simulink model "Particle_swarm_based_PV_MPPT"  (R2017a)
(part 3 of 6)

      mask TypeOptions ModuleName: User-defined | 1Soltech 1STH-215-P | 1Soltech 1STH-220-P | 1Soltech 1STH-225-P | 1Soltech 1STH-230-P | 1Soltech 1STH-235-WH | 1Soltech 1STH-240-WH | 1Soltech 1STH-245-WH | 1Soltech 1STH-FRL-4H-245-M60-BLK | 1Soltech 1STH-250-WH | 1Soltech 1STH-FRL-4H-250-M60-BLK | 1Soltech 1STH-FRL-4H-255-M60-BLK | 1Soltech 1STH-FRL-4H-260-M60-BLK | 1Soltech 1STH-335-WH | 1Soltech 1STH-340-WH | 1Soltech 1STH-345-WH | 1Soltech 1STH-350-WH | A10Green Technology A10J-S72-175 | A10Green Technology A10J-S72-180 | A10Green Technology A10J-S72-185 | A10Green Technology A10J-M60-220 | A10Green Technology A10J-M60-225 | A10Green Technology A10J-M60-230 | A10Green Technology A10J-M60-235 | A10Green Technology A10J-M60-240 | A2Peak Power POWER ON P220-6x10 | Aavid Solar ASMS-165P | Aavid Solar ASMS-180M | Aavid Solar ASMS-185M | Aavid Solar ASMS-220P | Aavid Solar ASMS-225M | Aavid Solar ASMS-230P | Aavid Solar ASMS-235M | Aavid Solar ASMS-270P | Aavid Thermalloy ASMP-175M | Aavid Thermalloy ASMP-180M | AblyTek 5MN6C175-A0 | AblyTek 5MN6C180-A0 | AblyTek 5MN6C185-A0 | AblyTek 6PN6A220-A0 | AblyTek 6PN6A225-A0 | AblyTek 6PN6A230-A0 | AblyTek 6PN6A235-A0 | AblyTek 6PN6A240-A0 | AccuSolar Power ASP610-B230 | Advance Solar Hydro Wind Power API-150 | Advance Solar Hydro Wind Power API-160 | Advance Solar Hydro Wind Power API-165 | Advance Solar Hydro Wind Power API-170 | Advance Solar Hydro Wind Power API-175 | Advance Solar Hydro Wind Power API-180 | Advance Solar Hydro Wind Power API156P-200 | Advance Solar Hydro Wind Power API156P-210 | Advance Solar Hydro Wind Power API156P-220 | Advance Solar Hydro Wind Power API156P-230 | Advanced Renewable Energy AREi-210W-M6-G | Advanced Renewable Energy AREi-215W-M6-G | Advanced Renewable Energy AREi-220W-M6-G | Advanced Renewable Energy AREi-225W-M6-G | Advanced Renewable Energy AREi-230W-M6-G | aleo solar S16.165 | aleo solar S16.170 | aleo solar S16.175 | aleo solar S16.180 | aleo solar S16.185 | aleo solar A18.210 | Aleo Solar A18U210 ulr | aleo solar S18.210 | Aleo Solar S18U210 ulr | aleo solar A18.215 | Aleo Solar A18U215 ulr | aleo solar S18.215 | Aleo Solar S18U215 ulr | aleo solar A18.220 | Aleo Solar A18U220 ulr | aleo solar S18.220 | Aleo Solar S18U220 ulr | aleo solar A18.225 | Aleo Solar A18U225 ulr | aleo solar S18.225 | Aleo Solar S18U225 ulr | aleo solar A18.230 | Aleo Solar A18U230 ulr | aleo solar A79.230 | Aleo Solar A79U230 ulr | aleo solar S18.230 | Aleo Solar S18U230 ulr | aleo solar S79.230 | Aleo Solar S79U230 ulr | aleo solar A18.235 | Aleo Solar A18U235 ulr | aleo solar A79.235 | Aleo Solar A79U235 ulr | aleo solar S18.235 | Aleo Solar S18U235 ulr | Aleo Solar S19U235 ulr | aleo solar S79.235 | Aleo Solar S79U235 ulr | aleo solar A18.240 | Aleo Solar A18U240 ulr | aleo solar A79.240 | Aleo Solar A79U240 ulr | aleo solar S18.240 | Aleo Solar S18U240 | Aleo Solar S18U240 ulr | Aleo Solar S19U240 ulr | aleo solar S79.240 | Aleo Solar S79U240 ulr | aleo solar A18.245 | Aleo Solar A18U245 ulr | aleo solar A79.245 | Aleo Solar A79U245 ulr | aleo solar S18.245 | Aleo Solar S18U245 | Aleo Solar S18U245 ulr | Aleo Solar S19U245 ulr | aleo solar S79.245 | Aleo Solar S79U245 ulr | aleo solar A79.250 | Aleo Solar A79U250 ulr | Aleo Solar S18U250 | Aleo Solar S19H250 | Aleo Solar S19U250 ulr | aleo solar S79.250 | Aleo Solar S79U250 | Aleo Solar S79U250 ulr | Aleo Solar S18U255 | Aleo Solar S19H255 | Aleo Solar S19U255 ulr | Aleo Solar S79U255 | Aleo Solar S18U260 | Aleo Solar S19H260 | Aleo Solar S79U260 | Aleo Solar S19H265 | Aleo Solar S79U265 | Aleo Solar S19H270 | Aleo Solar S79U270 | alfasolar alfasolar P6L60-220 | alfasolar alfasolar P6L60-225 | alfasolar alfasolar P6L60-230 | alfasolar alfasolar P6L60-235 | alfasolar alfasolar M6L60-240 | alfasolar alfasolar P6L60-240 | alfasolar alfasolar M6L60-245 | alfasolar alfasolar P6L60-245 | alfasolar alfasolar M6L60-250 | alfasolar alfasolar P6L60-250 | alfasolar alfasolar M6L60-255 | alfasolar alfasolar M6L60-260 | alfasolar alfasolar M6L60-265 | Alps Technology ATI-S572-175 | Alps Technology ATI-S572-180 | Alps Technology ATI-S572-185 | Alps Technology ATI-M660-220 | Alps Technology ATI-M660-225 | Alps Technology ATI-M660-230 | Alps Technology ATI-M660-235 | Alps Technology ATI-M660-240 | American Choice Solar ACS-215-P | American Choice Solar ACS-220-P | American Choice Solar ACS-225-P | American Choice Solar ACS-230-P | American Choice Solar ACS-235-M | American Choice Solar ACS-240-M | American Choice Solar ACS-245-M | American Choice Solar ACS-250-M | American Choice Solar ACS-335-M | American Solar Wholesale ASW-175M | American Solar Wholesale ASW-180M | American Solar Wholesale ASW-185M | American Solar Wholesale ASW-215P | American Solar Wholesale ASW-220P | American Solar Wholesale ASW-225M | American Solar Wholesale ASW-225P | American Solar Wholesale ASW-230M | American Solar Wholesale ASW-230P | American Solar Wholesale ASW-235M | American Solar Wholesale ASW-235P | American Solar Wholesale ASW-240M-60 | American Solar Wholesale ASW-245M | American Solar Wholesale ASW-250P | American Solar Wholesale ASW-260M | American Solar Wholesale ASW-260P | American Solar Wholesale ASW-265M | American Solar Wholesale ASW-270M | American Solar Wholesale ASW-270P | American Solar Wholesale ASW-275M | American Solar Wholesale ASW-280M | American Value SM240-5M | American Value SM245-5M | American Value SM250-5M | American Value SM255-5M | American Value SM260-5M | Andalay Solar ST_165_1_DC0_0_B | Andalay Solar ST165-1 | Andalay Solar ST_170_1_DC0_0_B | Andalay Solar ST170-1 | Andalay Solar ST_175_1_DC0_0_B | Andalay Solar ST175-1 | Andalay Solar ST-175-1AC1-A-A | Andalay Solar ST-175-1AC3-B-A | Andalay Solar KC180-1 | Andalay Solar ST_180_1_DC0_0_B | Andalay Solar ST180-1 | Andalay Solar ST_185_1_DC0_0_B | Andalay Solar ST-185-1 | Andalay Solar ST-185-1AC1-A-A | Andalay Solar ST-185-1AC1-A-B | Andalay Solar ST-185-1AC3-B-A | Andalay Solar ST-185-1AC3-B-B | Andalay Solar ST_190_1_DC0_0_B | Andalay Solar ST-190-1AC1-A-B | Andalay Solar ST-190-1AC3-B-B | Andalay Solar ST_195_1_DC0_0_B | Andalay Solar ST-195-1AC1-A-B | Andalay Solar ST-195-1AC3-B-B | Andalay Solar KC205-1 | Andalay Solar KC210-1 | Andalay Solar LW-230-1-AC0-D-B | Andalay Solar LW-230-1-AC1-A-B | Andalay Solar LW-230-1-AC2-D-B | Andalay Solar LW-230-1-AC3-B-B | Andalay Solar LW-230-1-DC0-0-B | Andalay Solar LW-230-1-DC0-0-BL | Andalay Solar LW-230-1-DC1-0-B | Andalay Solar LW-235-1-AC0-D-B | Andalay Solar LW-235-1-AC1-A-B | Andalay Solar LW-235-1-AC2-D-B | Andalay Solar LW-235-1-AC3-B-B | Andalay Solar LW-235-1-DC0-0-B | Andalay Solar LW-235-1-DC0-0-BL | Andalay Solar LW-235-1-DC1-0-B | Andalay Solar LW-240-1-AC0-D-B | Andalay Solar LW-240-1-AC1-A-B | Andalay Solar LW-240-1-AC2-D-B | Andalay Solar LW-240-1-AC3-B-B | Andalay Solar LW-240-1-DC0-0-B | Andalay Solar LW-240-1-DC0-0-BL | Andalay Solar LW-240-1-DC1-0-B | Andalay Solar TW-240-1-AC2-D-B | Andalay Solar TW-240-1-DC4-0-B | Andalay Solar TW-245-1-AC2-D-B | Andalay Solar TW-245-1-DC4-0-B | Andalay Solar TW-250-1-AC2-D-B | Andalay Solar TW-250-1-DC4-0-B | Andalay Solar ST_260_1_DC0_0_B | Andalay Solar ST_270_1_DC0_0_B | Andalay Solar ST_280_1_DC0_0_B | Andalay Solar ST_290_1_DC0_0_B | Anji Dasol Solar Energy Science & Technology DS-A4-210 | Anji Dasol Solar Energy Science & Technology DS-A4-215 | Anji Dasol Solar Energy Science & Technology DS-A4-220 | Anji Dasol Solar Energy Science & Technology DS-A4-225 | Anji Dasol Solar Energy Science & Technology DS-A4-230 | Anji Technology AJP-S572-175 | Anji Technology AJP-S572-180 | Anji Technology AJP-S572-185 | Anji Technology AJP-M660-220 | Anji Technology AJP-M660-225 | Anji Technology AJP-M660-230 | Anji Technology AJP-M660-235 | Anji Technology AJP-M660-240 | Anji Technology AJP-M660-245 | Anji Technology AJP-M660-250 | Antaris Solar AS P 230 | Antaris Solar SM-230PC8 | Antaris Solar SM-235PC8 | Antaris Solar SM-240PC8 | Antaris Solar SM-245PC8 | Antaris Solar SM-250PC8 | Antaris Solar SM-275PC8 | Antaris Solar SM-280PC8 | Antaris Solar SM-285PC8 | Antaris Solar SM-290PC8 | Antaris Solar SM-295PC8 | Apollo Solar Energy ASEC-120G6M | Apollo Solar Energy ASEC-125G6M | Apollo Solar Energy ASEC-125G6S | Apollo Solar Energy ASEC-130G6M | Apollo Solar Energy ASEC-130G6S | Apollo Solar Energy ASEC-135G6M | Apollo Solar Energy ASEC-135G6S | Apollo Solar Energy ASEC-140G6M | Apollo Solar Energy ASEC-140G6S | Apollo Solar Energy ASEC-145G6M49 | Apollo Solar Energy ASEC-145G6S49 | Apollo Solar Energy ASEC-150G6M49 | Apollo Solar Energy ASEC-150G6S49 | Apollo Solar Energy ASEC-155G6M49 | Apollo Solar Energy ASEC-155G6S49 | Apollo Solar Energy ASEC-175G6M | Apollo Solar Energy ASEC-175G6S | Apollo Solar Energy ASEC-180G6M | Apollo Solar Energy ASEC-180G6S | Apollo Solar Energy ASEC-185G6M | Apollo Solar Energy ASEC-185G6S | Apollo Solar Energy ASEC-190G6M | Apollo Solar Energy ASEC-190G6M68 | Apollo Solar Energy ASEC-190G6S | Apollo Solar Energy ASEC-190G6S68 | Apollo Solar Energy ASEC-195G6M | Apollo Solar Energy ASEC-195G6M68 | Apollo Solar Energy ASEC-195G6S | Apollo Solar Energy ASEC-195G6S68 | Apollo Solar Energy ASEC-200G6M | Apollo Solar Energy ASEC-200G6M68 | Apollo Solar Energy ASEC-200G6S | Apollo Solar Energy ASEC-200G6S68 | Apollo Solar Energy ASEC-205G6M | Apollo Solar Energy ASEC-205G6M68 | Apollo Solar Energy ASEC-205G6S | Apollo Solar Energy ASEC-205G6S68 | Apollo Solar Energy ASEC-210G6M | Apollo Solar Energy ASEC-210G6M68 | Apollo Solar Energy ASEC-210G6S | Apollo Solar Energy ASEC-210G6S68 | Apollo Solar Energy ASEC-215G6M | Apollo Solar Energy ASEC-215G6M68 | Apollo Solar Energy ASEC-215G6M69 | Apollo Solar Energy ASEC-215G6S | Apollo Solar Energy ASEC-215G6S68 | Apollo Solar Energy ASEC-215G6S69 | Apollo Solar Energy ASEC-220G6M | Apollo Solar Energy ASEC-220G6M68 | Apollo Solar Energy ASEC-220G6M69 | Apollo Solar Energy ASEC-220G6S | Apollo Solar Energy ASEC-220G6S68 | Apollo Solar Energy ASEC-220G6S69 | Apollo Solar Energy ASEC-225G6M | Apollo Solar Energy ASEC-225G6M69 | Apollo Solar Energy ASEC-225G6S | Apollo Solar Energy ASEC-225G6S69 | Apollo Solar Energy ASEC-230G6M | Apollo Solar Energy ASEC-230G6M69 | Apollo Solar Energy ASEC-230G6S | Apollo Solar Energy ASEC-230G6S69 | Apollo Solar Energy ASEC-235G6M | Apollo Solar Energy ASEC-235G6M69 | Apollo Solar Energy ASEC-235G6S | Apollo Solar Energy ASEC-235G6S69 | Apollo Solar Energy ASEC-240G6M69 | Apollo Solar Energy ASEC-240G6M6A | Apollo Solar Energy ASEC-240G6S69 | Apollo Solar Energy ASEC-240G6S6A | Apollo Solar Energy ASEC-245G6M | Apollo Solar Energy ASEC-245G6M69 | Apollo Solar Energy ASEC-245G6M6A | Apollo Solar Energy ASEC-245G6S69 | Apollo Solar Energy ASEC-245G6S6A | Apollo Solar Energy ASEC-250G6M | Apollo Solar Energy ASEC-250G6M6A | Apollo Solar Energy ASEC-250G6M6B | Apollo Solar Energy ASEC-250G6S6A | Apollo Solar Energy ASEC-250G6S6B | Apollo Solar Energy ASEC-255G6M | Apollo Solar Energy ASEC-255G6M6A | Apollo Solar Energy ASEC-255G6M6B | Apollo Solar Energy ASEC-255G6S | Apollo Solar Energy ASEC-255G6S6A | Apollo Solar Energy ASEC-255G6S6B | Apollo Solar Energy ASEC-260G6M | Apollo Solar Energy ASEC-260G6M6A | Apollo Solar Energy ASEC-260G6M6B | Apollo Solar Energy ASEC-260G6S | Apollo Solar Energy ASEC-260G6S6A | Apollo Solar Energy ASEC-260G6S6B | Apollo Solar Energy ASEC-265G6M | Apollo Solar Energy ASEC-265G6M6A | Apollo Solar Energy ASEC-265G6M6B | Apollo Solar Energy ASEC-265G6S | Apollo Solar Energy ASEC-265G6S6A | Apollo Solar Energy ASEC-265G6S6B | Apollo Solar Energy ASEC-270G6M | Apollo Solar Energy ASEC-270G6M6A | Apollo Solar Energy ASEC-270G6M6B | Apollo Solar Energy ASEC-270G6S | Apollo Solar Energy ASEC-270G6S6A | Apollo Solar Energy ASEC-270G6S6B | Apollo Solar Energy ASEC-275G6M | Apollo Solar Energy ASEC-275G6M6B | Apollo Solar Energy ASEC-275G6S | Apollo Solar Energy ASEC-275G6S6B | Apollo Solar Energy ASEC-280G6M | Apollo Solar Energy ASEC-280G6M6B | Apollo Solar Energy ASEC-280G6S | Apollo Solar Energy ASEC-280G6S6B | Apollo Solar Energy ASEC-285G6M | Apollo Solar Energy ASEC-285G6M6B | Apollo Solar Energy ASEC-285G6S | Apollo Solar Energy ASEC-285G6S6B | Apollo Solar Energy ASEC-290G6M | Apollo Solar Energy ASEC-290G6M6B | Apollo Solar Energy ASEC-290G6S | Apollo Solar Energy ASEC-290G6S6B | Apollo Solar Energy ASEC-295G6M | Apollo Solar Energy ASEC-295G6M6B | Apollo Solar Energy ASEC-295G6S | Apollo Solar Energy ASEC-295G6S6B | Apollo Solar Energy ASEC-300G6M | Apollo Solar Energy ASEC-300G6S | Apollo Solar Energy ASEC-305G6M | Apollo Solar Energy ASEC-305G6S | Apollo Solar Energy ASEC-310G6M | Apollo Solar Energy ASEC-310G6S | Apollo Solar Energy ASEC-315G6M | Apollo Solar Energy ASEC-315G6S | Apollo Solar Energy ASEC-320G6M | Apollo Solar Energy ASEC-320G6S | Apollo Solar Energy ASEC-325G6M | Apollo Solar Energy ASEC-325G6S | APOS Energy AP130 | APOS Energy AP135 | APOS Energy AS135 | APOS Energy AP140 | APOS Energy AS140 | APOS Energy AS145 | APOS Energy AP175 | APOS Energy AP180 | APOS Energy AS180 | APOS Energy AP185 | APOS Energy AS185 | APOS Energy AP190 | APOS Energy AS190 | APOS Energy AP195 | APOS Energy AS195 | APOS Energy AP 200M | APOS Energy AP200 | APOS Energy AS200 | APOS Energy AP 205M | APOS Energy AP205 | APOS Energy AS205 | APOS Energy AP 210M | APOS Energy AP210 | APOS Energy AS210 | APOS Energy AP 215M | APOS Energy AP215 | APOS Energy AS215 | APOS Energy AP 220M | APOS Energy AP220 | APOS Energy AS220 | APOS Energy AP 225M | APOS Energy AP225 | APOS Energy AS225 | APOS Energy AP 230M | APOS Energy AP230 | APOS Energy AS230 | APOS Energy AP 235M | APOS Energy AS235 | APOS Energy AP 240M | APOS Energy AS240 | Applied Quantum Technology AQT125MA-160W | Applied Quantum Technology AQT125MA-165W | Applied Quantum Technology AQT125MA-170W | Applied Quantum Technology AQT125MA-175W | Applied Quantum Technology AQT125MA-180W | Applied Quantum Technology AQT156PA-190W | Applied Quantum Technology AQT156PA-195W | Applied Quantum Technology AQT156PA-200W | Applied Quantum Technology AQT156PA-205W | Applied Quantum Technology AQT156PA-210W | Applied Quantum Technology AQT156PA-215W | Applied Quantum Technology AQT156PA-220W | Applied Quantum Technology AQT156PA-225W | Applied Quantum Technology AQT156PA-230W | Armageddon Energy SolarClover Dual Module | ASUN Energy ASM190PCA0G101 | ASUN Energy ASM195PCA0G101 | ASUN Energy ASM200PCA0G101 | ASUN Energy ASM205PCA0G101 | ASUN Energy ASM210PCA0G101 | Atersa (Aplicaciones Tecnicas de la Energia) A-225P | Atersa (Aplicaciones Tecnicas de la Energia) A-230P | Atersa (Aplicaciones Tecnicas de la Energia) A-235P | Atersa (Aplicaciones Tecnicas de la Energia) A-240P | Atersa (Aplicaciones Tecnicas de la Energia) A-245P | Atersa (Aplicaciones Tecnicas de la Energia) A-250P | Atersa (Aplicaciones Tecnicas de la Energia) A-275P | Atersa (Aplicaciones Tecnicas de la Energia) A-280P | Atersa (Aplicaciones Tecnicas de la Energia) A-285P | Atersa (Aplicaciones Tecnicas de la Energia) A-290P | Atersa (Aplicaciones Tecnicas de la Energia) A-295P | Atersa (Aplicaciones Tecnicas de la Energia) A-300P | Atlantis Energy Systems SS125LM | Atlantis Energy Systems SS156LM | Atlantis Energy Systems TS125LM | Atlantis Energy Systems TSG156LM | Atlantis Energy Systems TSG156GM | Atlantis Energy Systems SS125GM | Atlantis Energy Systems SS156GM | Atlantis Energy Systems TS125GM | Atlantis Energy AES-SS-100-C | Atlantis Energy AES-SS-100-W | AU Optronics PM180M00.0_170 | AU Optronics PM180M00.0_175 | AU Optronics PM180M00.0_180 | AU Optronics PM200M00_190 | AU Optronics PM200M00_195 | AU Optronics PM200M00_200 | AU Optronics PM200M00_205 | AU Optronics PM200M00_210 | AU Optronics PM220P00_215 | AU Optronics PM220P02.0_215 | AU Optronics PM220P00.4_220 | AU Optronics PM220P00_220 | AU Optronics PM220P01.0_220 | AU Optronics PM220P02.0_220 | AU Optronics PM220P00.4_225 | AU Optronics PM220P00_225 | AU Optronics PM220P01.0_225 | AU Optronics PM220P02.0_225 | AU Optronics PM245P00_225 | AU Optronics PM220P00.4_230 | AU Optronics PM220P00_230 | AU Optronics PM220P01.0_230 | AU Optronics PM220P02.0_230 | AU Optronics PM240P00_230 | AU Optronics PM245P00_230 | AU Optronics PM245P01_230 | AU Optronics PM060PA0_235 | AU Optronics PM060PA1_235 | AU Optronics PM060PA2_235 | AU Optronics PM220P00.4_235 | AU Optronics PM220P00_235 | AU Optronics PM220P01.0_235 | AU Optronics PM240P00_235 | AU Optronics PM240PA0_235 | AU Optronics PM245P00_235 | AU Optronics PM245P01_235 | AU Optronics PM245PA0_235 | AU Optronics PM245PA1_235 | AU Optronics PM245PA2_235 | AU Optronics PM060MA0_240 | AU Optronics PM060MA1_240 | AU Optronics PM060MA2_240 | AU Optronics PM060PA0_240 | AU Optronics PM060PA1_240 | AU Optronics PM060PA2_240 | AU Optronics PM220P01.0_240 | AU Optronics PM240P00_240 | AU Optronics PM240PA0_240 | AU Optronics PM245P00_240 | AU Optronics PM245P01_240 | AU Optronics PM245PA0_240 | AU Optronics PM245PA1_240 | AU Optronics PM245PA2_240 | AU Optronics PM250M00_240 | AU Optronics PM250M02_240 | AU Optronics PM250MA0_240 | AU Optronics PM250MA1_240 | AU Optronics PM250MA2_240 | AU Optronics PM060MA0_245 | AU Optronics PM060MA1_245 | AU Optronics PM060MA2_245 | AU Optronics PM060PA0_245 | AU Optronics PM060PA1_245 | AU Optronics PM060PA2_245 | AU Optronics PM240P00_245 | AU Optronics PM240PA0_245 | AU Optronics PM245P00_245 | AU Optronics PM245P01_245 | AU Optronics PM245PA0_245 | AU Optronics PM245PA1_245 | AU Optronics PM245PA2_245 | AU Optronics PM250M00_245 | AU Optronics PM250MA0_245 | AU Optronics PM250MA1_245 | AU Optronics PM250MA2_245 | AU Optronics PM060MA0_250 | AU Optronics PM060MA1_250 | AU Optronics PM060MA2_250 | AU Optronics PM060PA0_250 | AU Optronics PM060PA1_250 | AU Optronics PM060PA2_250 | AU Optronics PM245P00_250 | AU Optronics PM245P01_250 | AU Optronics PM245PA0_250 | AU Optronics PM245PA1_250 | AU Optronics PM245PA2_250 | AU Optronics PM250M00_250 | AU Optronics PM250M01_250 | AU Optronics PM250MA0_250 | AU Optronics PM250MA1_250 | AU Optronics PM250MA2_250 | AU Optronics PM060MA0_255 | AU Optronics PM060MA1_255 | AU Optronics PM060MA2_255 | AU Optronics PM060PA0_255 | AU Optronics PM060PA1_255 | AU Optronics PM060PA2_255 | AU Optronics PM245P00_255 | AU Optronics PM245P01_255 | AU Optronics PM245PA0_255 | AU Optronics PM245PA1_255 | AU Optronics PM245PA2_255 | AU Optronics PM250M00_255 | AU Optronics PM250M01_255 | AU Optronics PM250MA0_255 | AU Optronics PM250MA1_255 | AU Optronics PM250MA2_255 | AU Optronics PM060MA0_260 | AU Optronics PM060MA1_260 | AU Optronics PM060MA2_260 | AU Optronics PM060PA0_260 | AU Optronics PM060PA1_260 | AU Optronics PM060PA2_260 | AU Optronics PM245P00_260 | AU Optronics PM245P01_260 | AU Optronics PM245PA0_260 | AU Optronics PM245PA1_260 | AU Optronics PM245PA2_260 | AU Optronics PM250M00_260 | AU Optronics PM250M01_260 | AU Optronics PM250MA0_260 | AU Optronics PM250MA1_260 | AU Optronics PM250MA2_260 | AU Optronics PM060MA0_265 | AU Optronics PM060MA1_265 | AU Optronics PM060MA2_265 | AU Optronics PM250M00_265 | AU Optronics PM250M01_265 | AU Optronics PM250MA0_265 | AU Optronics PM250MA1_265 | AU Optronics PM250MA2_265 | AU Optronics PM060MA0_270 | AU Optronics PM060MA1_270 | AU Optronics PM060MA2_270 | AU Optronics PM250M00_270 | AU Optronics PM250M01_270 | AU Optronics PM250MA0_270 | AU Optronics PM250MA1_270 | AU Optronics PM250MA2_270 | AU Optronics PM300P00_270 | AU Optronics PM300P00_275 | AU Optronics PM300P00_280 | AU Optronics PM300P00_285 | AU Optronics PM300P00_290 | AU Optronics PM300P00_295 | AU Optronics PM300P00_300 | AU Optronics PM300P00_305 | AU Optronics PM300P00_310 | AU Optronics PM300P00_315 | Auria Solar M115000 | Auria Solar M120000 | Auria Solar M125000 | Auxin Solar AXN-P6T160 | Auxin Solar AXN-M5T165 | Auxin Solar AXN-P6T165 | Auxin Solar AXN-M5T170 | Auxin Solar AXN-P6T170 | Auxin Solar AXN-M5T175 | Auxin Solar AXN-P6T175 | Auxin Solar AXN-M5T180 | Auxin Solar AXN-P6T180 | Auxin Solar AXN-P6T190 | Auxin Solar AXN-P6T195 | Auxin Solar AXN-P6T200 | Auxin Solar AXN-P6T205 | Auxin Solar AXN-P6T210 | Auxin Solar AXN-P6T215 | Auxin Solar AXN-P6T220 | Auxin Solar AXN-P6T225 | Auxin Solar AXN-P6T230 | Auxin Solar AXN-P6T235 | Auxin Solar AXN-P6T240 | Auxin Solar AXN-P6T245 | Auxin Solar AXN-P6T250 | Auxin Solar AXN-P6T255 | Auxin Solar AXN-P6T260 | Auxin Solar AXN-P6T265 | Auxin Solar AXN-P6T270 | Auxin Solar AXN-P6T275 | Auxin Solar AXN-P6T280 | Auxin Solar AXN-P6T285 | Avancis PowerMax 100 FB | Avancis PowerMax STRONG 115 | Avancis PowerMax 120FB | Avancis PowerMax STRONG 120 | Avancis PowerMax STRONG 125 | Avancis PowerMax STRONG 130 | Axitec AC-190M-125-72S | Axitec AC-195M-125-72S | Axitec AC-200M-125-72S | Axitec AC-230M-156-60S | Axitec AC-235M-156-60S | Axitec AC-235P-156-60B | Axitec AC-235P-156-60S | Axitec AC-240M-156-60S | Axitec AC-240P-156-60B | Axitec AC-240P-156-60S | Axitec AC-245M-156-60S | Axitec AC-245P-156-60S | Axitec AC-250M-156-60S | Axitec AC-250P-156-60S | AXITEC AC-255M-156-60S | AXITEC AC-255P-156-60S | AXITEC AC-260M-156-60S | AXITEC AC-260P-156-60S | AXITEC AC-265M-156-60S | Axitec AC-285M-156-72S | Axitec AC-285P-156-72S | Axitec AC-290M-156-72S | Axitec AC-290P-156-72S | Axitec AC-295M-156-72S | Axitec AC-295P-156-72S | Axitec AC-300M-156-72S | AXITEC AC-300P-156-72S | AXITEC AC-305M-156-72S | AXITEC AC-305P-156-72S | AXITEC AC-310M-156-72S | AXITEC AC-310P-156-72S | AXITEC AC-315M-156-72S | AxunTek Solar Energy AA963450170 | AxunTek Solar Energy AA963450175 | AxunTek Solar Energy AA963450180 | Axuntek Solar Energy AR931200132 | Axuntek Solar Energy AR931200134 | Axuntek Solar Energy AR931200136 | Axuntek Solar Energy AR931200138 | Bangkok Solar BS-52 | Baoding Tianwei Solarfilms TWSE-aSi-80W-1 | Baoding Tianwei Solarfilms TWSF-aSi-80W-1 | Baoding Tianwei Solarfilms TWSF-W-aSi-80W-1 | Baoding Tianwei Solarfilms TWSE-aSi-85W-1 | Baoding Tianwei Solarfilms TWSF-aSi-85W-1 | Baoding Tianwei Solarfilms TWSF-W-aSi-85W-1 | Baoding Tianwei Solarfilms TWSE-aSi-90W-1 | Baoding Tianwei Solarfilms TWSF-aSi-90W-1 | Baoding Tianwei Solarfilms TWSF-W-aSi-90W-1 | Baoding Tianwei Solarfilms TWSE-aSi-95W-1 | Baoding Tianwei Solarfilms TWSF-aSi-95W-1 | Baoding Tianwei Solarfilms TWSF-W-aSi-95W-1 | Baoding Tianwei Solarfilms TWSE-aSi-100W-1 | Baoding Tianwei Solarfilms TWSF-aSi-100W-1 | Baoding Tianwei Solarfilms TWSF-W-aSi-100W-1 | Beijing Zhongkexin Electronics Equipment ZKX-180D-24 | Beijing Zhongkexin Electronics Equipment ZKX-185D-24 | Beijing Zhongkexin Electronics Equipment ZKX-190D-24 | Beijing Zhongkexin Electronics Equipment ZKX-265P-24 | Beijing Zhongkexin Electronics Equipment ZKX-270P-24 | Beijing Zhongkexin Electronics Equipment ZKX-275P-24 | Beijing Zhongkexin Electronics Equipment ZKX-280P-24 | Beijing Zhongkexin Electronics Equipment ZKX-285P-24 | BIPV BIPV050-S11 | BIPV BIPV050-T11 | BIPV BIPV050-T16 | BIPV BIPV050-T86 | BIPV BIPV052-S11 | BIPV BIPV052-S16 | BIPV BIPV052-S86 | BIPV BIPV052-T11 | BIPV BIPV052-T16 | BIPV BIPV052-T86 | BIPV BIPV054-S11 | BIPV BIPV054-S16 | BIPV BIPV054-S86 | BIPV BIPV054-T16 | BIPV BIPV054-T86 | BJ Penn BJP240M-B | BJ Penn BJP245M-B | BJ Penn BJP245M-Bv | BJ Penn BJP245S-B | BJ Penn BJP250M-B | BJ Penn BJP250M-Bv | BJ Penn BJP250S-B | BJ Penn BJP255M-B | BJ Penn BJP255M-Bv | BJ Penn BJP255S-B | BJ Penn BJP260M-Bv | BJ Penn BJP265M-Bv | BJ Penn BJP270M-A | BJ Penn BJP275M-A | BJ Penn BJP280M-A | BJ Penn BJP285M-A | BJ Penn BJP285M-Av | BJ Penn BJP290M-A | BJ Penn BJP290M-Av | BJ Penn BJP295M-A | BJ Penn BJP295M-Av | BJ Penn BJP300M-A | BJ Penn BJP300M-Av | BJ Penn BJP305M-A | BJ Penn BJP305M-Av | BJ Penn BJP310M-Av | BJ Penn BJP315M-Av | Bluechip Energy AP-215MK | Bluechip Energy AP-220MK | Bluechip Energy AP-220PK | Bluechip Energy AP-225MK | Bluechip Energy AP-225PK | Bluechip Energy AP-230MK | Bluechip Energy AP-230PK | Bluechip Energy AP-235MK | Bluechip Energy AP-235PK | Bluechip Energy AP-240MK | Bluechip Energy AP-240PK | Bluechip Energy AP-245MK | Bluechip Energy ASP-390M | Bluechip Energy ASP-395M | Bluechip Energy ASP-400M | Bluechip Energy ASP-405M | Bluechip Energy ASP-410M | Bosch Solar Energy c-Si M 60-225-16 | Bosch Solar Energy c-Si M 60 NA30117 230W | Bosch Solar Energy c-Si M 60-230-16 | Bosch Solar Energy c-Si M 60 NA30117 235W | Bosch Solar Energy c-Si M 60-235-16 | Bosch Solar Energy c-Si M 60 NA30117 240W | Bosch Solar Energy c-Si M 60-240-16 | Bosch Solar Energy c-Si M60 NA30119-240Wp | Bosch Solar Energy c-Si M 60 NA30117 245W | Bosch Solar Energy c-Si M60 NA30119-245Wp | Bosch Solar Energy c-Si M60 NA42117 245W | Bosch Solar Energy c-Si M60 NA30119-250Wp | Bosch Solar Energy c-Si M60 NA42117 250W | Bosch Solar Energy c-Si M60 NA30119-255Wp | Bosch Solar Energy c-Si M60 NA42117 255W | Bosch Solar Energy c-Si P 72 NA21126 275Wp | Bosch Solar Energy c-Si P 72 NA22126 275Wp | Bosch Solar Energy c-Si P 72 NA21126 280Wp | Bosch Solar Energy c-Si P 72 NA22126 280Wp | Bosch Solar Energy c-Si P 72 NA21126 285Wp | Bosch Solar Energy c-Si P 72 NA22126 285Wp | Bosch Solar Energy c-Si M 72 NA41126 290Wp | Bosch Solar Energy c-Si P 72 NA21126 290Wp | Bosch Solar Energy c-Si P 72 NA22126 290Wp | Bosch Solar Energy c-Si M 72 NA41126 295Wp | Bosch Solar Energy c-Si P 72 NA21126 295Wp | Bosch Solar Energy c-Si P 72 NA22126 295Wp | Bosch Solar Energy c-Si M 72 NA41126 300Wp | Bosch Solar Energy c-Si M 72 NA41126 305Wp | Bosch Solar Thin Film um-Si plus 105 | Bosch Solar Thin Film um-Si plus 110 | Bosch Solar Thin Film um-Si plus 115 | BP Solar BP365TS | BP Solar BP170B | BP Solar BP3170B | BP Solar BP3170N | BP Solar BP3170N_Q | BP Solar BP3170T | BP Solar BP4170B | BP Solar BP175B | BP Solar BP175I | BP Solar BP3175B | BP Solar BP3175N | BP Solar BP3175N_Q | BP Solar BP3175T | BP Solar BP4175B | BP Solar BP4175T | BP Solar BP3180N | BP Solar BP3180N_Q | BP Solar BP4180B | BP Solar BP4180T | BP Solar BP4185B | BP Solar BP4185T | BP Solar BP4190T | BP Solar SX3190B | BP Solar SX3190N | BP Solar SX3190W | BP Solar SX3195B | BP Solar SX3195N | BP Solar SX3195W | BP Solar SX3200B | BP Solar SX3200N | BP Solar SX3200W | BP Solar BP3210N | BP Solar BP3210T | BP Solar BP3215B | BP Solar BP3220N | BP Solar BP3220Q | BP Solar BP3220T | BP Solar BP3225B | BP Solar BP3225N | BP Solar BP3225Q | BP Solar BP3225T | BP Solar BP3230N | BP Solar BP3230Q | BP Solar BP3230T | BP Solar BP3235N | BP Solar BP3235Q | BP Solar BP3235T | BP Solar BP3237T | BP Solar BP3270T | BP Solar BP3280T | Brightwatts BWI-72-P175 | Brightwatts BWI-60-M190 | Brightwatts BI-156-200W | Brightwatts BWI-60-M200 | Brightwatts BWI-60-M220 | Brightwatts BWI-96-M220 | Brightwatts BWI-60-M225 | Brightwatts BWI-96-M225 | Brightwatts BWI-60-M230 | Brightwatts BWI-96-M230 | BYD (Huizhou) Battery BYD 120P6-18 | BYD (Huizhou) Battery BYD 125P6-18 | BYD (Huizhou) Battery BYD 130P6-18 | BYD (Huizhou) Battery BYD 135P6-18 | BYD (Huizhou) Battery BYD 140P6-18 | BYD (Huizhou) Battery BYD 200P6-30 | BYD (Huizhou) Battery BYD 205P6-30 | BYD (Huizhou) Battery BYD 210P6-30 | BYD (Huizhou) Battery BYD 215P6-30 | BYD (Huizhou) Battery BYD 220P6-30 | BYD (Huizhou) Battery BYD 220P6A-30 | BYD (Huizhou) Battery BYD 225P6-30 | BYD (Huizhou) Battery BYD 225P6A-30 | BYD (Huizhou) Battery BYD 230P6-30 | BYD (Huizhou) Battery BYD 230P6A-30 | BYD (Huizhou) Battery BYD 235P6-30 | BYD (Huizhou) Battery BYD 235P6A-30 | BYD (Huizhou) Battery BYD 235P6C-30 | BYD (Huizhou) Battery BYD 240P6-30 | BYD (Huizhou) Battery BYD 240P6-36 | BYD (Huizhou) Battery BYD 240P6A-30 | BYD (Huizhou) Battery BYD 240P6C-30 | BYD (Huizhou) Battery BYD 245P6-36 | BYD (Huizhou) Battery BYD 245P6A-30 | BYD (Huizhou) Battery BYD 245P6C-30 | BYD (Huizhou) Battery BYD 250P6-36 | BYD (Huizhou) Battery BYD 250P6A-30 | BYD (Huizhou) Battery BYD 250P6C-30 | BYD (Huizhou) Battery BYD 255P6-36 | BYD (Huizhou) Battery BYD 255P6C-30 | BYD (Huizhou) Battery BYD 260P6-36 | BYD (Huizhou) Battery BYD 260P6A-36 | BYD (Huizhou) Battery BYD 265P6-36 | BYD (Huizhou) Battery BYD 265P6A-36 | BYD (Huizhou) Battery BYD 270P6-36 | BYD (Huizhou) Battery BYD 270P6A-36 | BYD (Huizhou) Battery BYD 275P6-36 | BYD (Huizhou) Battery BYD 275P6A-36 | BYD (Huizhou) Battery BYD 280P6-36 | BYD (Huizhou) Battery BYD 280P6A-36 | BYD (Huizhou) Battery BYD 280P6C-36 | BYD (Huizhou) Battery BYD 285P6-36 | BYD (Huizhou) Battery BYD 285P6A-36 | BYD (Huizhou) Battery BYD 285P6C-36 | BYD (Huizhou) Battery BYD 290P6A-36 | BYD (Huizhou) Battery BYD 290P6C-36 | BYD (Huizhou) Battery BYD 295P6A-36 | BYD (Huizhou) Battery BYD 295P6C-36 | BYD (Huizhou) Battery BYD 300P6A-36 | BYD (Huizhou) Battery BYD 300P6C-36 | BYD (Huizhou) Battery BYD 305P6C-36 | CA Solar MS-150M | CA Solar MS-155M | CA Solar MS-160M | CA Solar MS-165M | CA Solar MS-170M | CA Solar MS-175M | CA Solar MS-180M | Canadian Solar CS5C-80M | Canadian Solar CS5C-90M | Canadian Solar CS5T-130M | Canadian Solar CS5T-135M | Canadian Solar CS5T-140M | Canadian Solar CS6C-140P | Canadian Solar CS5T-145M | Canadian Solar CS6C-145P | Canadian Solar CS5A-150M | Canadian Solar CS5T-150M | Canadian Solar CS6A-150P | Canadian Solar CS6A-150PE | Canadian Solar CS5A-155M | Canadian Solar CS6A-155P | Canadian Solar CS6A-155PE | Canadian Solar CS5A-160M | Canadian Solar CS5A-160MX | Canadian Solar CS6A-160P | Canadian Solar CS6A-160PE | Canadian Solar CS6P-160PE | Canadian Solar CS5A-165M | Canadian Solar CS5A-165MX | Canadian Solar CS6A-165P | Canadian Solar CS6P-165PE | Canadian Solar CS5A-170M | Canadian Solar CS5A-170MX | Canadian Solar CS6A-170P | Canadian Solar CS6P-170PE | Canadian Solar CS5A-175M | Canadian Solar CS5A-175MX | Canadian Solar CS6A-175P | Canadian Solar CS6P-175PE | Canadian Solar CS5A-180M | Canadian Solar CS5A-180MX | Canadian Solar CS6A-180P | Canadian Solar CS6P-180P | Canadian Solar CS6P-180PE | Canadian Solar CS5A-185M | Canadian Solar CS5A-185MX | Canadian Solar CS6A-185P | Canadian Solar CS6P-185P | Canadian Solar CS6P-185PE | Canadian Solar CS5A-190M | Canadian Solar CS5A-190MX | Canadian Solar CS6A-190MM | Canadian Solar CS6A-190P | Canadian Solar CS6P-190P | Canadian Solar CS6P-190PE | Canadian Solar CS5A-195M | Canadian Solar CS5A-195MX | Canadian Solar CS5P-195M | Canadian Solar CS6A-195MM | Canadian Solar CS6P-195P | Canadian Solar CS6P-195PE | Canadian Solar CS5A-200M | Canadian Solar CS5P-200M | Canadian Solar CS6A-200MM | Canadian Solar CS6P-200P | Canadian Solar CS6P-200PE | Canadian Solar CS6P-200PX | Canadian Solar CS5P-205M | Canadian Solar CS6A-205MM | Canadian Solar CS6P-205M | Canadian Solar CS6P-205P | Canadian Solar CS6P-205PE | Canadian Solar CS6P-205PX | Canadian Solar CS5P-210M | Canadian Solar CS6A-210MM | Canadian Solar CS6P-210M | Canadian Solar CS6P-210P | Canadian Solar CS6P-210PE | Canadian Solar CS6P-210PX | Canadian Solar CS5P-215M | Canadian Solar CS6P-215M | Canadian Solar CS6P-215P | Canadian Solar CS6P-215PE | Canadian Solar CS6P-215PX | Canadian Solar CS5P-220M | Canadian Solar CS5P-220P | Canadian Solar CS6P-220M | Canadian Solar CS6P-220P | Canadian Solar CS6P-220PE | Canadian Solar CS6P-220PX | Canadian Solar CS5P-225M | Canadian Solar CS5P-225P | Canadian Solar CS6P-225P | Canadian Solar CS6P-225PE | Canadian Solar CS6P-225PX | Canadian Solar CS5P-230M | Canadian Solar CS5P-230P | Canadian Solar CS6P-230M | Canadian Solar CS6P-230MX | Canadian Solar CS6P-230P | Canadian Solar CS6P-230PE | Canadian Solar CS6P-230PT | Canadian Solar CS6P-230PX | Canadian Solar CS5P-235M | Canadian Solar CS5P-235P | Canadian Solar CS6P-235M | Canadian Solar CS6P-235MX | Canadian Solar CS6P-235P | Canadian Solar CS6P-235PM | Canadian Solar CS6P-235PT | Canadian Solar CS6P-235PX | Canadian Solar CS5P-240M | Canadian Solar CS5P-240P | Canadian Solar CS6P-240M | Canadian Solar CS6P-240MX | Canadian Solar CS6P-240P | Canadian Solar CS6P-240PM | Canadian Solar CS6P-240PT | Canadian Solar CS6P-240PX | Canadian Solar CS5P-245M | Canadian Solar CS6P-245M | Canadian Solar CS6P-245M-EA | Canadian Solar CS6P-245MM | Canadian Solar CS6P-245MX | Canadian Solar CS6P-245P | Canadian Solar CS6P-245P-EA | Canadian Solar CS6P-245PM | Canadian Solar CS6P-245PT | Canadian Solar CS6P-245PX | Canadian Solar CS5P-250M | Canadian Solar CS6P-250M | Canadian Solar CS6P-250M-EA | Canadian Solar CS6P-250MM | Canadian Solar CS6P-250MX | Canadian Solar CS6P-250P | Canadian Solar CS6P-250P-EA | Canadian Solar CS6P-250PM | Canadian Solar CS6P-250PT | Canadian Solar CS6P-250PX | Canadian Solar CS5P-255M | Canadian Solar CS6P-255M | Canadian Solar CS6P-255M-EA | Canadian Solar CS6P-255MM | Canadian Solar CS6P-255P | Canadian Solar CS6P-255PM | Canadian Solar CS6X-255M | Canadian Solar CS6X-255P | Canadian Solar CS6P-260M | Canadian Solar CS6P-260M-EA | Canadian Solar CS6P-260MM | Canadian Solar CS6X-260M | Canadian Solar CS6X-260P | Canadian Solar CS6P-265M | Canadian Solar CS6P-265MM | Canadian Solar CS6X-265M | Canadian Solar CS6X-265P | Canadian Solar CS6X-270M | Canadian Solar CS6X-270P | Canadian Solar CS6X-275M | Canadian Solar CS6X-275P | Canadian Solar CS6X-280M | Canadian Solar CS6X-280P | Canadian Solar CS6X-285M | Canadian Solar CS6X-285P | Canadian Solar CS6X-290M | Canadian Solar CS6X-290P | Canadian Solar CS6X-295M | Canadian Solar CS6X-295P | Canadian Solar CS6X-300M | Canadian Solar CS6X-300P | Canadian Solar CS6X-305M | Canadian Solar CS6X-305P | Canadian Solar CS6X-310M | Canadian Solar CS6X-310P | Centennial Solar CS200 | Centrosolar America E165 | Centrosolar America E170 | Centrosolar America E175 | Centrosolar America E180 | Centrosolar America E185 | Centrosolar America E195 | Centrosolar America D200 | Centrosolar America E200 | Centrosolar America E205 | Centrosolar America D210 | Centrosolar America E210 | Centrosolar America D220 | Centrosolar America E220 | Centrosolar America E220B | Centrosolar America E225 | Centrosolar America E225B | Centrosolar America EP6 225 BW | Centrosolar America EP6 225 SW | Centrosolar America K225 | Centrosolar America K225B | Centrosolar America D230 | Centrosolar America E230 | Centrosolar America E230B | Centrosolar America E230BWZ | Centrosolar America E230SWZ | Centrosolar America EP6 230 BW | Centrosolar America EP6 230 SW | Centrosolar America K230 | Centrosolar America K230B | Centrosolar America BP6235BB | Centrosolar America BP6-235BW | Centrosolar America BP6235SW | Centrosolar America E235 | Centrosolar America E235B | Centrosolar America E235BWZ | Centrosolar America E235SWZ | Centrosolar America EP6 235 BW | Centrosolar America EP6 235 SW | Centrosolar America K235 | Centrosolar America K235B | Centrosolar America BP6-240BB | Centrosolar America BP6-240BW | Centrosolar America BP6-240SW | Centrosolar America E240 | Centrosolar America E240B | Centrosolar America E240BWZ | Centrosolar America E240SWZ | Centrosolar America EP6 240 BW | Centrosolar America EP6 240 SW | Centrosolar America BP6-245BB | Centrosolar America BP6-245BW | Centrosolar America BP6-245SW | Centrosolar America E245 | Centrosolar America E245B | Centrosolar America EP6 245 BW | Centrosolar America EP6 245 SW | Centrosolar America BP6-250BB | Centrosolar America BP6-250BW | Centrosolar America BP6-250SW | Centrosolar America E250 | Centrosolar America E250B | Centrosolar America EP6 250BW | Centrosolar America EP6 250SW | Centrosolar America BP6-255BB | Centrosolar America BP6-255BW | Centrosolar America BP6-255SW | Centrosolar America EP6 255BW | Centrosolar America EP6 255SW | Centrosolar America BP6-260BB | Centrosolar America BP6-260BW | Centrosolar America BP6-260SW | Centrosolar America E260 | Centrosolar America EP6 260BW | Centrosolar America EP6 260SW | Centrosolar America BP6-265BB | Centrosolar America BP6-265BW | Centrosolar America BP6-265SW | Centrosolar America E265 | Centrosolar America E265B | Centrosolar America EP6 265BW | Centrosolar America EP6 265SW | Centrosolar America BP6-270BB | Centrosolar America BP6-270BW | Centrosolar America BP6-270SW | Centrosolar America E270 | Centrosolar America E270B | Centrosolar America E275 | Centrosolar America E275B | Centrosolar America EP7 275 BW | Centrosolar America EP7 275 SW | Centrosolar America E280 | Centrosolar America E280B | Centrosolar America EP7 280 BW | Centrosolar America EP7 280 SW | Centrosolar America BP7-285SW | Centrosolar America E285 | Centrosolar America E285B | Centrosolar America EP7 285 BW | Centrosolar America EP7 285 SW | Centrosolar America BP7-290SW | Centrosolar America E290 | Centrosolar America E290B | Centrosolar America EP7 290 BW | Centrosolar America EP7 290 SW | Centrosolar America BP7-295SW | Centrosolar America E295 | Centrosolar America E295B | Centrosolar America EP7 295 BW | Centrosolar America EP7 295 SW | Centrosolar America BP7-300SW | Centrosolar America E300 | Centrosolar America E300B | Centrosolar America BP7-305BW | Centrosolar America BP7-305SW | Centrosolar America E305 | Centrosolar America E305B | Centrosolar America BP7-310BW | Centrosolar America BP7-310SW | Centrosolar America BP7-315BW | Centrosolar America BP7-315SW | Centrosolar America BP7-320BW | Centrosolar America BP7-320SW | Centrosolar Canada SP6 220SW | Centrosolar Canada SP6 225SW | Centrosolar Canada SP6 230SW | Centrosolar Canada SP6 235SW | Centrosolar Canada SP6 240SW | Centrosolar Canada SP6 245SW | Centrosolar Canada SP6 250SW | Centrosolar Canada SP6 255SW | Centrosolar Canada SP7 265SW | Centrosolar Canada SP7 270SW | Centrosolar Canada SP7 275SW | Centrosolar Canada SP7 280SW | Centrosolar Canada SP7 285SW | CentroSolar Sonnenstromfabrik CP6230BW | CentroSolar Sonnenstromfabrik CP6230SW | CentroSolar Sonnenstromfabrik CP6235BW | CentroSolar Sonnenstromfabrik CP6235SW | CentroSolar Sonnenstromfabrik CP6240BW | CentroSolar Sonnenstromfabrik CP6240SW | CertainTeed Apollo | CertainTeed APOLLO TILE-B | CertainTeed APOLLO TILE-G | CertainTeed Apollo II | Changzhou Almaden SEAP60-230 | Changzhou Almaden SEAP60-235 | Changzhou Almaden SEAP60-240 | Changzhou Almaden SEAP60-245 | Changzhou Almaden SEAP60-250 | Changzhou Almaden SEAP60-255 | Changzhou Almaden SEAP60-260 | Changzhou Almaden SEAP72-280 | Changzhou Almaden SEAP72-285 | Changzhou Almaden SEAP72-290 | Changzhou Almaden SEAP72-295 | Changzhou Almaden SEAP72-300 | Changzhou Almaden SEAP72-305 | Changzhou Eging Photovoltaic Technology EGM-150 | Changzhou Eging Photovoltaic Technology EGM-155 | Changzhou Eging Photovoltaic Technology EGM-160 | Changzhou Eging Photovoltaic Technology EGM-165 | Changzhou Eging Photovoltaic Technology EG-170P48-C | Changzhou Eging Photovoltaic Technology EGM-170 | Changzhou Eging Photovoltaic Technology EG-175P48-C | Changzhou Eging Photovoltaic Technology EGM-175 | Changzhou Eging Photovoltaic Technology EG-180M48-C | Changzhou Eging Photovoltaic Technology EG-180P48-C | Changzhou Eging Photovoltaic Technology EGM-180 | Changzhou Eging Photovoltaic Technology EG-185M48-C | Changzhou Eging Photovoltaic Technology EGM-185 | Changzhou Eging Photovoltaic Technology EG-190M48-C | Changzhou Eging Photovoltaic Technology EG-190P54-C | Changzhou Eging Photovoltaic Technology EGM-190 | Changzhou Eging Photovoltaic Technology EG-195P54-C | Changzhou Eging Photovoltaic Technology EG-200P54-C | Changzhou Eging Photovoltaic Technology EG-205M54-C | Changzhou Eging Photovoltaic Technology EG-205P54-C | Changzhou Eging Photovoltaic Technology EG-210M54-C | Changzhou Eging Photovoltaic Technology EG-210P54-C | Changzhou Eging Photovoltaic Technology EG-210P60-C | Changzhou Eging Photovoltaic Technology EG-215M54-C | Changzhou Eging Photovoltaic Technology EG-215P60-C | Changzhou Eging Photovoltaic Technology EG-220P60-C | Changzhou Eging Photovoltaic Technology EG-225M60-C | Changzhou Eging Photovoltaic Technology EG-225P60-C | Changzhou Eging Photovoltaic Technology EG-230M60-C | Changzhou Eging Photovoltaic Technology EG-230P60-C | Changzhou Eging Photovoltaic Technology EG-235M60-C | Changzhou Eging Photovoltaic Technology EG-240M72-C | Changzhou Eging Photovoltaic Technology EG-245M72-C | Changzhou Eging Photovoltaic Technology EG-255P72-C | Changzhou Eging Photovoltaic Technology EG-260P72-C | Changzhou Eging Photovoltaic Technology EG-265M72-C | Changzhou Eging Photovoltaic Technology EG-265P72-C | Changzhou Eging Photovoltaic Technology EG-270M72-C | Changzhou Eging Photovoltaic Technology EG-270P72-C | Changzhou Eging Photovoltaic Technology EG-275M72-C | Changzhou Eging Photovoltaic Technology EG-275P72-C | Changzhou Eging Photovoltaic Technology EG-280M72-C | Changzhou Eging Photovoltaic Technology EG-280P72-C | Changzhou Eging Photovoltaic Technology EG-285M72-C | Changzhou Nesl Solartech DJ-165D | Changzhou Nesl Solartech DJ-170D | Changzhou Nesl Solartech DJ-175D | Changzhou Nesl Solartech DJ-180D | Changzhou Nesl Solartech DJ-185D | Changzhou Nesl Solartech DJ-190D | Changzhou Nesl Solartech DJ-195D | Changzhou Nesl Solartech DJ-200D | Changzhou Nesl Solartech DJ-200P | Changzhou Nesl Solartech DJ-210P | Changzhou Nesl Solartech DJ-220P | Changzhou Nesl Solartech DJ-230P | Changzhou Nesl Solartech DJ-230P-ST15 | Changzhou Nesl Solartech DJ-235P | Changzhou Nesl Solartech DJ-235P-ST15 | Changzhou Nesl Solartech DJ-240DA-C | Changzhou Nesl Solartech DJ-240DA-C-ST15 | Changzhou Nesl Solartech DJ-240P | Changzhou Nesl Solartech DJ-240PA | Changzhou Nesl Solartech DJ-240P-ST15 | Changzhou Nesl Solartech DJ-245DA-C | Changzhou Nesl Solartech DJ-245DA-C-ST15 | Changzhou Nesl Solartech DJ-250DA-C | Changzhou Nesl Solartech DJ-250DA-C-ST15 | Changzhou Nesl Solartech DJ-250P | Changzhou Nesl Solartech DJ-255D-C | Changzhou Nesl Solartech DJ-255D-C-ST15 | Changzhou Nesl Solartech DJ-260P | Changzhou Nesl Solartech DJ-270P | Changzhou Nesl Solartech DJ-280P | Changzhou Nesl Solartech DJ-285P | Changzhou Nesl Solartech DJ-290D-C | Changzhou Nesl Solartech DJ-290P | Changzhou Nesl Solartech DJ-295D-C | Changzhou Nesl Solartech DJ-295P | Changzhou Nesl Solartech DJ-300D-C | Changzhou Nesl Solartech DJ-300P | Changzhou Nesl Solartech DJ-305D-C | Changzhou Nesl Solartech DJ-310D-C | Chi Mei Energy CSSU-100A | Chi Mei Energy CSSU-100B | China Sunergy (Nanjing) CSUN170-72M | China Sunergy (Nanjing) CSUN175-72M | China Sunergy (Nanjing) SST175-72M | China Sunergy (Nanjing) CSUN180-72M | China Sunergy (Nanjing) SST180-72M | China Sunergy (Nanjing) CSUN185-72M | China Sunergy (Nanjing) SST185-72M | China Sunergy (Nanjing) CSUN190-72M | China Sunergy (Nanjing) SST190-72M | China Sunergy (Nanjing) CSUN215-54M-BB | China Sunergy (Nanjing) SST215-54M | China Sunergy (Nanjing) SST215-54M-BB | China Sunergy (Nanjing) CSUN220-54M-BB | China Sunergy (Nanjing) SST220-54M | China Sunergy (Nanjing) SST220-54M-BB | China Sunergy (Nanjing) SST220-60M | China Sunergy (Nanjing) SST220-60P | China Sunergy (Nanjing) CSUN225-54M-BB | China Sunergy (Nanjing) SST225-54M | China Sunergy (Nanjing) SST225-54M-BB | China Sunergy (Nanjing) SST225-60M | China Sunergy (Nanjing) SST225-60P | China Sunergy (Nanjing) SST230-60M | China Sunergy (Nanjing) SST230-60P | China Sunergy (Nanjing) CSUN235-60M-BB | China Sunergy (Nanjing) CSUN235-60P-BW | China Sunergy (Nanjing) SST235-60M | China Sunergy (Nanjing) SST235-60M-BB | China Sunergy (Nanjing) SST235-60P | China Sunergy (Nanjing) SST235-60P-BW | China Sunergy (Nanjing) CSUN240-54M | China Sunergy (Nanjing) CSUN240-60M-BB | China Sunergy (Nanjing) CSUN240-60P-BW | China Sunergy (Nanjing) SST240-54M | China Sunergy (Nanjing) SST240-60M | China Sunergy (Nanjing) SST240-60M-BB | China Sunergy (Nanjing) SST240-60P | China Sunergy (Nanjing) SST240-60P-BW | China Sunergy (Nanjing) CSUN245-60M | China Sunergy (Nanjing) CSUN245-60M-BB | China Sunergy (Nanjing) CSUN245-60M-BW | China Sunergy (Nanjing) CSUN245-60P | China Sunergy (Nanjing) CSUN245-60P-BW | China Sunergy (Nanjing) SST245-60M | China Sunergy (Nanjing) SST245-60M-BB | China Sunergy (Nanjing) SST245-60M-BW | China Sunergy (Nanjing) SST245-60P | China Sunergy (Nanjing) SST245-60P-BW | China Sunergy (Nanjing) CSUN250-60M | China Sunergy (Nanjing) CSUN250-60M-BW | China Sunergy (Nanjing) CSUN250-60P | China Sunergy (Nanjing) CSUN250-60P-BW | China Sunergy (Nanjing) SST250-60M | China Sunergy (Nanjing) SST250-60M-BW | China Sunergy (Nanjing) SST250-60P | China Sunergy (Nanjing) SST250-60P-BW | China Sunergy (Nanjing) CSUN255-60M | China Sunergy (Nanjing) CSUN255-60M-BW | China Sunergy (Nanjing) CSUN255-60P | China Sunergy (Nanjing) CSUN255-60P-BW | China Sunergy (Nanjing) SST255-60M | China Sunergy (Nanjing) SST255-60M-BW | China Sunergy (Nanjing) SST255-60P | China Sunergy (Nanjing) SST255-60P-BW | China Sunergy (Nanjing) CSUN260-60M | China Sunergy (Nanjing) CSUN260-60M-BW | China Sunergy (Nanjing) CSUN260-60P | China Sunergy (Nanjing) SST260-60M | China Sunergy (Nanjing) SST260-60M-BW | China Sunergy (Nanjing) SST260-60P | China Sunergy (Nanjing) CSUN265-60M | China Sunergy (Nanjing) CSUN265-60M-BW | China Sunergy (Nanjing) SST265-60M | China Sunergy (Nanjing) SST265-60M-BW | China Sunergy (Nanjing) SST265-72M | China Sunergy (Nanjing) CSUN270-60M | China Sunergy (Nanjing) SST270-60M | China Sunergy (Nanjing) SST270-72M | China Sunergy (Nanjing) SST275-72M | China Sunergy (Nanjing) SST275-72P | China Sunergy (Nanjing) CSUN280-72M-BB | China Sunergy (Nanjing) CSUN280-72P | China Sunergy (Nanjing) SST280-72M | China Sunergy (Nanjing) SST280-72M-BB | China Sunergy (Nanjing) SST280-72P | China Sunergy (Nanjing) CSUN285-72M-BB | China Sunergy (Nanjing) SST285-72M | China Sunergy (Nanjing) SST285-72M-BB | China Sunergy (Nanjing) SST285-72P | China Sunergy (Nanjing) CSUN290-72M-BB | China Sunergy (Nanjing) SST290-72M | China Sunergy (Nanjing) SST290-72M-BB | China Sunergy (Nanjing) SST290-72P | China Sunergy (Nanjing) CSUN295-72M-BB | China Sunergy (Nanjing) SST295-72M | China Sunergy (Nanjing) SST295-72M-BB | China Sunergy (Nanjing) SST300-72M | China Sunergy (Nanjing) CSUN305-72M | China Sunergy (Nanjing) SST305-72M | China Sunergy (Nanjing) CSUN310-72M | China Sunergy (Nanjing) SST310-72M | China Sunergy (Nanjing) CSUN315-72M | China Sunergy (Nanjing) SST315-72M | China Sunergy (Nanjing) CSUN320-72M | China Sunergy (Nanjing) SST320-72M | China Sunergy CSUN215-54M | China Sunergy CSUN220-54M | China Sunergy CSUN220-60M | China Sunergy CSUN220-60P | China Sunergy CSUN225-54M | China Sunergy CSUN225-60M | China Sunergy CSUN225-60P | China Sunergy CSUN230-60M | China Sunergy CSUN230-60P | China Sunergy CSUN235-60M | China Sunergy CSUN240-60M | China Sunergy CSUN240-60P | China Sunergy CSUN245-60M | China Sunergy CSUN245-72M | China Sunergy CSUN250-60M | China Sunergy CSUN250-72M | China Sunergy CSUN265-72M | China Sunergy CSUN270-72M | China Sunergy CSUN275-72M | China Sunergy CSUN275-72P | China Sunergy CSUN280-72M | China Sunergy CSUN285-72M | China Sunergy CSUN285-72P | China Sunergy CSUN290-72M | China Sunergy CSUN290-72P | China Sunergy CSUN295-72M | China Sunergy CSUN300-72M | Chinalight Haoyu Photovoltaic Technology (Beijing) CLS165P | Chinalight Haoyu Photovoltaic Technology (Beijing) CLS170P | Chinalight Haoyu Photovoltaic Technology (Beijing) CLS175P | Chinalight Haoyu Photovoltaic Technology (Beijing) CLS180P | Chinalight Haoyu Photovoltaic Technology (Beijing) CLS185P | Chinalight Haoyu Photovoltaic Technology (Beijing) CLS190P | Chinalight Haoyu Photovoltaic Technology (Beijing) CLS215P | Chinalight Haoyu Photovoltaic Technology (Beijing) CLS220P | Chinalight Haoyu Photovoltaic Technology (Beijing) CLS-225P | Chinalight Haoyu Photovoltaic Technology (Beijing) CLS-230P | Chinalight Haoyu Photovoltaic Technology (Beijing) CLS-235P | Chinalight Haoyu Photovoltaic Technology (Beijing) CLS-240P | Chinalight Haoyu Photovoltaic Technology (Beijing) CLS-245P | Chinalight Haoyu Photovoltaic Technology (Beijing) CLS-250P | Chint Solar (Zhejiang) CHSM5001T-105 | Chint Solar (Zhejiang) CHSM5001T-110 | Chint Solar (Zhejiang) CHSM5001T-115 | Chint Solar (Zhejiang) CHSM5031T-125 | Chint Solar (Zhejiang) CHSM5031T-130 | Chint Solar (Zhejiang) CHSM5031T-135 | Chint Solar (Zhejiang) CHSM5612M-175 | Chint Solar (Zhejiang) CHSM5612M-180 | Chint Solar (Zhejiang) CHSM5612M(BL)-185 | Chint Solar (Zhejiang) CHSM5612M-185 | Chint Solar (Zhejiang) CHSM5612M(BL)-190 | Chint Solar (Zhejiang) CHSM5612M-190 | Chint Solar (Zhejiang) CHSM5612M(BL)-195 | Chint Solar (Zhejiang) CHSM5612M-195 | Chint Solar (Zhejiang) CHSM5612M(BL)-200 | Chint Solar (Zhejiang) CHSM5612M-200 | Chint Solar (Zhejiang) CHSM5612M-205 | Chint Solar (Zhejiang) CHSM5612M-210 | Chint Solar (Zhejiang) CHSM6609M-215 | Chint Solar (Zhejiang) CHSM6610P-215 | Chint Solar (Zhejiang) CHSM6609M-220 | Chint Solar (Zhejiang) CHSM6610M-220 | Chint Solar (Zhejiang) CHSM6610P-220 | Chint Solar (Zhejiang) CHSM6609M-225 | Chint Solar (Zhejiang) CHSM6610M-225 | Chint Solar (Zhejiang) CHSM6610P-225 | Chint Solar (Zhejiang) CHSM6609M-230 | Chint Solar (Zhejiang) CHSM6610M-230 | Chint Solar (Zhejiang) CHSM6610P-230 | Chint Solar (Zhejiang) CHSM6609M-235 | Chint Solar (Zhejiang) CHSM6610M-235 | Chint Solar (Zhejiang) CHSM6610P-235 | Chint Solar (Zhejiang) CHSM6609M-240 | Chint Solar (Zhejiang) CHSM6610M(BL)-240 | Chint Solar (Zhejiang) CHSM6610M-240 | Chint Solar (Zhejiang) CHSM6610P-240 | Chint Solar (Zhejiang) CHSM6610M(BL)-245 | Chint Solar (Zhejiang) CHSM6610M-245 | Chint Solar (Zhejiang) CHSM6610P-245 | Chint Solar (Zhejiang) CHSM6610M(BL)-250 | Chint Solar (Zhejiang) CHSM6610M-250 | Chint Solar (Zhejiang) CHSM6610P-250 | Chint Solar (Zhejiang) CHSM6610PR-250 | Chint Solar (Zhejiang) CHSM6610M(BL)-255 | Chint Solar (Zhejiang) CHSM6610M-255 | Chint Solar (Zhejiang) CHSM6610P-255 | Chint Solar (Zhejiang) CHSM6610PR-255 | Chint Solar (Zhejiang) CHSM6610M(BL)-260 | Chint Solar (Zhejiang) CHSM6610M-260 | Chint Solar (Zhejiang) CHSM6610P-260 | Chint Solar (Zhejiang) CHSM6610PR-260 | Chint Solar (Zhejiang) CHSM6612P-260 | Chint Solar (Zhejiang) CHSM6610M-265 | Chint Solar (Zhejiang) CHSM6610P-265 | Chint Solar (Zhejiang) CHSM6611P-265 | Chint Solar (Zhejiang) CHSM6612P-265 | Chint Solar (Zhejiang) CHSM6610M-270 | Chint Solar (Zhejiang) CHSM6611P-270 | Chint Solar (Zhejiang) CHSM6612P-270 | Chint Solar (Zhejiang) CHSM6610M-275 | Chint Solar (Zhejiang) CHSM6611P-275 | Chint Solar (Zhejiang) CHSM6612P-275 | Chint Solar (Zhejiang) CHSM6612PM-275 | Chint Solar (Zhejiang) CHSM6611P-280 | Chint Solar (Zhejiang) CHSM6612P-280 | Chint Solar (Zhejiang) CHSM6612PM-280 | Chint Solar (Zhejiang) CHSM6611P-285 | Chint Solar (Zhejiang) CHSM6612P-285 | Chint Solar (Zhejiang) CHSM6612PM-285 | Chint Solar (Zhejiang) CHSM6612P-290 | Chint Solar (Zhejiang) CHSM6612PM-290 | Chint Solar (Zhejiang) CHSM6612M-295 | Chint Solar (Zhejiang) CHSM6612P-295 | Chint Solar (Zhejiang) CHSM6612PM-295 | Chint Solar (Zhejiang) CHSM6612PR-295 | Chint Solar (Zhejiang) CHSM6612M-300 | Chint Solar (Zhejiang) CHSM6612P-300 | Chint Solar (Zhejiang) CHSM6612PR-300 | Chint Solar (Zhejiang) CHSM6612M-305 | Chint Solar (Zhejiang) CHSM6612P-305 | Chint Solar (Zhejiang) CHSM6612PR-305 | Chint Solar (Zhejiang) CHSM6612M-310 | Chint Solar (Zhejiang) CHSM6612P-310 | Chint Solar (Zhejiang) CHSM6612M-315 | Chint Solar (Zhejiang) CHSM6612M-320 | Chint Solar (Zhejiang) CHSM6612M-325 | Clean Source & Energy CSE115M-1 | Clean Source & Energy CSE120M-1 | Clean Source & Energy CSE125M-1 | Clean Source & Energy CSE150M-2 | Clean Source & Energy CSE155M-2 | Clean Source & Energy CSE160M-1 | Clean Source & Energy CSE160M-2 | Clean Source & Energy CSE165M-1 | Clean Source & Energy CSE165M-2 | Clean Source & Energy CSE170M-1 | Clean Source & Energy CSE170M-2 | Clean Source & Energy CSE175M-1 | Clean Source & Energy CSE175M-2 | Clean Source & Energy CSE180M-1 | Clean Source & Energy CSE180M-2 | Clean Source & Energy CSE180M-3 | Clean Source & Energy CSE185M-1 | Clean Source & Energy CSE185M-2 | Clean Source & Energy CSE190P-3 | Clean Source & Energy CSE195P-3 | Clean Source & Energy CSE200M-2 | Clean Source & Energy CSE200P-1 | Clean Source & Energy CSE200P-2 | Clean Source & Energy CSE200P-3 | Clean Source & Energy CSE205M-2 | Clean Source & Energy CSE205P-1 | Clean Source & Energy CSE205P-2 | Clean Source & Energy CSE205P-3 | Clean Source & Energy CSE210M-2 | Clean Source & Energy CSE210P-1 | Clean Source & Energy CSE210P-2 | Clean Source & Energy CSE215M-2 | Clean Source & Energy CSE215P-1 | Clean Source & Energy CSE215P-2 | Clean Source & Energy CSE220M-2 | Clean Source & Energy CSE220P-1 | Clean Source & Energy CSE220P-2 | Clean Source & Energy CSE220P-3 | Clean Source & Energy CSE220P-AS | Clean Source & Energy CSE225M-2 | Clean Source & Energy CSE225M-AS | Clean Source & Energy CSE225P-2 | Clean Source & Energy CSE225P-3 | Clean Source & Energy CSE230M-2 | Clean Source & Energy CSE230P-2 | Clean Source & Energy CSE230P-3 | Clean Source & Energy CSE230P-AS | Clean Source & Energy CSE235M-2 | Clean Source & Energy CSE235M-AS | Clean Source & Energy CSE240M-2 | Clean Source & Energy CSE250P-3 | Clean Source & Energy CSE255P-3 | Clean Source & Energy CSE270P-3 | Clean Source & Energy CSE275P-3 | Clean Source & Energy CSE280P-3 | CNBM International CNBM175SAb | CNBM International CNBM175SAb(Black) | CNBM International CNBM180SAb | CNBM International CNBM180SAb(Black) | CNBM International CNBM185SAb | CNBM International CNBM185SAb(Black) | CNBM International CNBM220PCe | CNBM International CNBM220PCe(Black) | CNBM International CNBM225PCe | CNBM International CNBM225PCe(Black) | CNBM International CNBM230PCe | CNBM International CNBM230PCe(Black) | CNBM International CNBM235PCe | CNBM International CNBM235PCe(Black) | CNBM International CNBM240PCe | CNBM International CNBM240PCe(Black) | CNPV Dongying Solar Power CNPV-170M | CNPV Dongying Solar Power CNPV-175M | CNPV Dongying Solar Power CNPV-180M | CNPV Dongying Solar Power CNPV-185M | CNPV Dongying Solar Power CNPV-190M | CNPV Dongying Solar Power CNPV-195M | CNPV Dongying Solar Power CNPV-200M | CNPV Dongying Solar Power CNPV-200P-54 | CNPV Dongying Solar Power CNPV-205M | CNPV Dongying Solar Power CNPV-205P-54 | CNPV Dongying Solar Power CNPV-210M-54 | CNPV Dongying Solar Power CNPV-210P-54 | CNPV Dongying Solar Power CNPV-215M-54 | CNPV Dongying Solar Power CNPV-215P-54 | CNPV Dongying Solar Power CNPV-220M-54 | CNPV Dongying Solar Power CNPV-220P-54 | CNPV Dongying Solar Power CNPV-225M-54 | CNPV Dongying Solar Power CNPV-225P | CNPV Dongying Solar Power CNPV-225P-54 | CNPV Dongying Solar Power CNPV-230M-54 | CNPV Dongying Solar Power CNPV-230P | CNPV Dongying Solar Power CNPV-230P-54 | CNPV Dongying Solar Power CNPV-235P | CNPV Dongying Solar Power CNPV-235P-54 | CNPV Dongying Solar Power CNPV-240M | CNPV Dongying Solar Power CNPV-240P | CNPV Dongying Solar Power CNPV-245M | CNPV Dongying Solar Power CNPV-245P | CNPV Dongying Solar Power CNPV-250M | CNPV Dongying Solar Power CNPV-250P | CNPV Dongying Solar Power CNPV-255M | CNPV Dongying Solar Power CNPV-255P | CNPV Dongying Solar Power CNPV-260M | CNPV Dongying Solar Power CNPV-260P | CNPV Dongying Solar Power CNPV-270P | CNPV Dongying Solar Power CNPV-275M | CNPV Dongying Solar Power CNPV-275P | CNPV Dongying Solar Power CNPV-280M | CNPV Dongying Solar Power CNPV-280P | CNPV Dongying Solar Power CNPV-285M | CNPV Dongying Solar Power CNPV-285P | CNPV Dongying Solar Power CNPV-290M | CNPV Dongying Solar Power CNPV-290P | CNPV Dongying Solar Power CNPV-295M | CNPV Dongying Solar Power CNPV-295P | CNPV Dongying Solar Power CNPV-300M | CNPV Dongying Solar Power CNPV-300P | CNPV Dongying Solar Power CNPV-305M | CNPV Dongying Solar Power CNPV-305P | CNPV Dongying Solar Power CNPV-310M | CNPV Dongying Solar Power CNPV-310P | CNPV Dongying Solar Power CNPV-315P | Colored Solar GCS-215-P60-C1-532 | Colored Solar GCS-220-P60-C2-653 | Colored Solar GCS-220-P60-C3-823 | Colored Solar GCS-220-P60-C4-433 | Colored Solar GCS-225-P60-C10-011 | Colored Solar GCS-225-P60-C11-012 | Colored Solar GCS-225-P60-C5-053 | Colored Solar GCS-225-P60-C6-033 | Colored Solar GCS-225-P60-C7-015 | Colored Solar GCS-225-P60-C8-018 | Colored Solar GCS-225-P60-C9-077 | Colored Solar GCS-230-M60-430 | Colored Solar GCS-245-M60-200 | Colored Solar GCS-250-M60-200 | Colored Solar GCS-335-M80-240 | Colored Solar GCS-340-M80-240 | Colored Solar GCS-350-M80-240 | Conergy Holding CONERGY ON 220-60 | Conergy Holding CONERGY ON 225-60 | Conergy Holding CONERGY ON 230-60 | Conergy Holding CONERGY ON 235-60 | Conergy Holding CONERGY ON 240-60 | Conergy Holding CONERGY ON 245-60 | Conergy Holding CONERGY ON 250-60 | Conergy Holding CONERGY ON 255-60 | Conergy Holding CONERGY ON 265P-72 | Conergy Holding CONERGY ON 270P-72 | Conergy Holding CONERGY ON 275P-72 | Conergy Holding CONERGY ON 280P-72 | Conergy Holding CONERGY ON 285P-72 | Conergy Solarmodule PowerPlus 215P | Conergy Solarmodule PowerPlus 220P | Conergy Solarmodule PowerPlus 225P | Conergy Conergy Black 170M | Conergy Conergy P 170M | Conergy Conergy Black 175M | Conergy Conergy P 175M | Conergy Conergy PH 175M | Conergy Conergy Black 180M | Conergy Conergy P 180M | Conergy Conergy Black 185M | Conergy Conergy P 185M | Conergy Conergy P 190P | Conergy Conergy P 195P | Conergy Conergy P 200P | Conergy Conergy P 205P | Conergy Conergy Black 210PA | Conergy Conergy P 210P | Conergy Conergy P 210PA | Conergy Conergy Black 215PA | Conergy Conergy P 215PA | Conergy Conergy Black 220PA | Conergy Conergy P 220PA | Conergy Conergy PH 220P | Conergy Conergy PM 220P | Conergy Conergy Black 225PA | Conergy Conergy P 225PA | Conergy Conergy PH 225P | Conergy Conergy PM 225P | Conergy Conergy Black 230PA | Conergy Conergy P 230PA | Conergy Conergy PH 230M | Conergy Conergy PH 230P | Conergy Conergy PM 230P | Conergy Conergy Black 235PA | Conergy Conergy P 235PA | Conergy Conergy PH 235M | Conergy Conergy PH 235P | Conergy Conergy PM 235P | Conergy Conergy PH 240M | Conergy Conergy PH 240M BL | Conergy Conergy PH 240P | Conergy Conergy PM 240P | Conergy Conergy PE 245P | Conergy Conergy PH 245M | Conergy Conergy PH 245M BL | Conergy Conergy PH 245P | Conergy Conergy PM 245P | Conergy Conergy PE 250P | Conergy Conergy PH 250M | Conergy Conergy PH 250M BL | Conergy Conergy PH 250P | Conergy Conergy PM 250P | Conergy Conergy PE 255P | Conergy Conergy PH 255M | Conergy Conergy PH 255M BL | Conergy Conergy PH 255P | Conergy Conergy PM 255P | Conergy Conergy PE 260P | Conergy Conergy PH 260M | Conergy Conergy PH 260P | Conergy Conergy PM 260P | Conergy Conergy PH 285P | Conergy Conergy PH 290P | Conergy Conergy PE 295P | Conergy Conergy PH 295P | Conergy Conergy PE 300P | Conergy Conergy PH 300P | Conergy Conergy PE 305P | Conergy Conergy PH 305P | Conergy Conergy PE 310P | Conergy Conergy PH 310P | Cosmos Energy SL195-18 | Cosmos Energy SL200-18 | Cosmos Energy SL205-18 | Cosmos Energy SL220-20 | Cosmos Energy SL225-20 | Cosmos Energy SL230-20 | CSG PVTech CSG160M2-24 | CSG PVTech CSG165M2-24 | CSG PVTech CSG170M2-24 | CSG PVTech CSG175M2-24 | CSG PVTech CSG175S1-36 | CSG PVTech CSG180M2-24 | CSG PVTech CSG180S1-36 | CSG PVTech CSG185S1 | CSG PVTech CSG190M2-27 | CSG PVTech CSG190S1 | CSG PVTech CSG195M2-27 | CSG PVTech CSG195S1 | CSG PVTech CSG200M2-27 | CSG PVTech CSG205M2-27 | CSG PVTech CSG220M2-30 | CSG PVTech CSG225M2-30 | CSG PVTech CSG230M2-30 | CSG PVTech CSG235M2 | CSG PVTech CSG235S2 | CSG PVTech CSG240M2 | CSG PVTech CSG240S2 | CSG PVTech CSG245M2 | CSG PVTech CSG245S2 | CSG PVTech CSG250M2-35 | CSG PVTech CSG250S2 | CSG PVTech CSG255M2-35 | CSG PVTech CSG255S2 | CSG PVTech CSG260M2-35 | CSG PVTech CSG260S2 | CSG PVTech CSG265M2-35 | CSG PVTech CSG265S2 | CSG PVTech CSG270M2-36 | CSG PVTech CSG275M2-36 | CSG PVTech CSG280M2-36 | CSG PVTech CSG285M2 | CSG PVTech CSG285S2 | CSG PVTech CSG290M2 | CSG PVTech CSG290S2 | CSG PVTech CSG295M2 | CSG PVTech CSG295S2 | CSG PVTech CSG300M2 | CSG PVTech CSG300S2 | CSG PVTech CSG305S2 | Cuantum Solar SUNPORT 275P | DJ Solar DJS175S125M-72 | DJ Solar DJS180S125M-72 | DJ Solar DJS-T180S6ST | DJ Solar DJS185S125M-72 | DJ Solar DJS-T185S6ST | DJ Solar DJS190S125M-72 | DJ Solar DJS-T190S6ST | DJ Solar DJS195S125M-72 | DJ Solar DJS-T195S648ST | DJ Solar DJS-T200S648ST | DJ Solar DJS-T205S6ST | DJ Solar DJS210S156P-60 | DJ Solar DJS-T210P6PT | DJ Solar DJS-T210S6ST | DJ Solar DJS215S156P-60 | DJ Solar DJS-T215P6PT | DJ Solar DJS-T215S6ST | DJ Solar DJS220S156P-60 | DJ Solar DJS-T220P6PT | DJ Solar DJS-T220S6ST | DJ Solar DJS225S156P-60 | DJ Solar DJS-T225P6PT | DJ Solar DJS-T225S654ST | DJ Solar DJS230S156P-60 | DJ Solar DJS-T230P6PT | DJ Solar DJS235S156P-60 | DJ Solar DJS-T235S6ST | DJ Solar DJS-TU235PT | DJ Solar DJS240S156P-60 | DJ Solar DJS-T240P6PT | DJ Solar DJS-T240PT | DJ Solar DJS-T240S6ST | DJ Solar DJS-T250P6PT | DJ Solar DJS-T245P660PT | DJ Solar DJS-T245P6PT | DJ Solar DJS-T245S6ST | DJ Solar DJS-T250P660PT | DJ Solar DJS-T250ST | DJ Solar DJS-T255P666PT | DJ Solar DJS-T255P6PT | DJ Solar DJS-T260P666PT | DJ Solar DJS-T260P6PT | DJ Solar DJS-T260S6ST | DJ Solar DJS-T265P666PT | DJ Solar DJS-T265P6PT | DJ Solar DJS-T265S666ST | DJ Solar DJS-T270P666PT | DJ Solar DJS-T270P6PT | DJ Solar DJS-T270S666ST | DJ Solar DJS-T275P6PT | DJ Solar DJS-T275S666ST | DJ Solar DJS-T280P6PT | DJ Solar DJS-T280S6ST | DJ Solar DJS-T285P6PT | DJ Solar DJS-T285S6ST | DJ Solar DJS-T290P672PT | DJ Solar DJS-T290S6ST | DJ Solar DJS-T295P672PT | DJ Solar DJS-T295S6ST | DJ Solar DJS-T300P672PT | DJ Solar DJS-T300S6ST | DJ Solar DJS-T305S6ST | Dmsolar DM160M2-24 | Dmsolar DM-M160 | Dmsolar DM165M2-24 | Dmsolar DM170M2-24 | Dmsolar DM-M170 | Dmsolar DM175M2-24 | Dmsolar DM175S1-36 | Dmsolar DM180M2-24 | Dmsolar DM180S1-36 | Dmsolar DM-M180 | Dmsolar DM190M2-27 | Dmsolar DM195M2-27 | Dmsolar DM200M2-27 | Dmsolar DM-P200 | Dmsolar DM205M2-27 | Dmsolar DM-P210 | Dmsolar DM220M2-30 | Dmsolar DM-M220 | Dmsolar DM-P220 | Dmsolar DM225M2-30 | Dmsolar DM230M2-30 | Dmsolar DM-M230 | Dmsolar DM-P230 | Dmsolar DM-M240 | Dmsolar DM250M2-35 | Dmsolar DM255M2-35 | Dmsolar DM260M2-35 | Dmsolar DM265M2-35 | Dmsolar DM270M2-36 | Dmsolar DM275M2-36 | Dmsolar DM280M2-36 | Dongfang Electric (Yixing) MAGI MGSM-235-60 | Dongfang Electric (Yixing) MAGI MGSM-240-60 | Dongfang Electric (Yixing) MAGI MGSM-245-60 | Dongfang Electric (Yixing) MAGI MGSM-250-60 | Dongfang Electric (Yixing) MAGI MGSM-255-60 | Dongfang Electric (Yixing) MAGI MGSM-285-72 | Dongfang Electric (Yixing) MAGI MGSM-290-72 | Dongfang Electric (Yixing) MAGI MGSM-295-72 | Dongfang Electric (Yixing) MAGI MGSM-300-72 | Dongfang Electric (Yixing) MAGI MGSM-305-72 | Dongfang Electric (Yixing) MAGI MGSM-310-72 | Dongfang Electric (Yixing) MAGI MGSM-315-72 | Dow Chemical DPS-09-1000 | Dow Chemical DPS-10-1000 | Dow Chemical DPS-11-1000 | Dow Chemical DPS-12-1000 | Dow Chemical DPS-12.5-1000 | Dow Chemical DPS-13-1000 | Du Pont Apollo DA095-A2 | Du Pont Apollo DA095-A6 | Du Pont Apollo DA100-A2 | Du Pont Apollo DA100-A6 | Du Pont Apollo DA102-A6 | Du Pont Apollo DA105-A2 | Du Pont Apollo DA105-A6 | Du Pont Apollo DA130-C2 | Du Pont Apollo DA133-C2 | Du Pont Apollo DA136-C2 | DuraComm DCS-6P-36-130 | DuraComm DCS-6P-36-135 | DuraComm DCS-6P-36-140 | DuraComm DCS-6P-36-145 | DuraComm DCS-6P-36-150 | DuraComm DCS-6P-48-175 | DuraComm DCS-6P-48-180 | DuraComm DCS-6P-48-185 | DuraComm DCS-6P-48-190 | DuraComm DCS-6P-48-195 | DuraComm DCS-6P-48-200 | DuraComm DCS-6P-54-200 | DuraComm DCS-6P-54-205 | DuraComm DCS-6P-54-210 | DuraComm DCS-6P-54-215 | DuraComm DCS-6P-54-220 | DuraComm DCS-6P-60-220 | DuraComm DCS-6P-54-225 | DuraComm DCS-6P-60-225 | DuraComm DCS-6P-54-230 | DuraComm DCS-6P-60-230 | DuraComm DCS-6P-60-235 | DuraComm DCS-6P-60-240 | DuraComm DCS-6P-60-245 | DuraComm DCS-6P-60-250 | DuraComm DCS-6P-60-255 | DuraComm DCS-6P-72-265 | DuraComm DCS-6P-72-270 | DuraComm DCS-6P-72-275 | DuraComm DCS-6P-72-280 | DuraComm DCS-6P-72-285 | DuraComm DCS-6P-72-290 | DuraComm DCS-6P-72-295 | DuraComm DCS-6P-72-300 | DuraComm DCS-6P-72-305 | E&H EHS3-228 | E&H EHS3-230 | E&H EHS3-233 | E&H EHS3-235 | E&H EHS3-238 | E&H EHS3-240 | E&H EHS3-243 | E&H EHS3-245 | E&H EHS3-248 | E&H EHS3-250 | Eclipsall Energy NRG60-230M-BK | Eclipsall Energy NRG60-235M-BK | Eclipsall Energy NRG60-240M | Eclipsall Energy NRG60-240M-BK | Eclipsall Energy NRG60-240P | Eclipsall Energy NRG60-245M | Eclipsall Energy NRG60-245M-BK | Eclipsall Energy NRG60-245P | Eclipsall Energy NRG60-250M | Eclipsall Energy NRG60-250M-BK | Eclipsall Energy NRG60-250P | Eclipsall Energy NRG60-255M | Eclipsall Energy NRG60-255P | Eclipsall Energy NRG60-260M | Eclipsall Energy NRG72-290M | Eclipsall Energy NRG72-290P | Eclipsall Energy NRG72-295M | Eclipsall Energy NRG72-295P | Eclipsall Energy NRG72-300M | Eclipsall Energy NRG72-300P | Eclipsall Energy NRG72-305M | Eclipsall Energy NRG72-305P | Eclipsall Energy NRG72-310M | Eclipsall Energy NRG72-310P | Eclipsall Energy NRG72-315M | Eclipsall Energy NRG72-320M | Econess Energy EN125M-72-185 | Econess Energy EN125M-72-190 | Econess Energy EN125M-72-195 | Econess Energy EN125M-72-200 | Econess Energy EN156M-60-235 | Econess Energy EN156P-60-235 | Econess Energy EN156M-60-240 | Econess Energy EN156P-60-240 | Econess Energy EN125M-96-245 | Econess Energy EN156M-60-245 | Econess Energy EN156P-60-245 | Econess Energy EN125M-96-250 | Econess Energy EN156M-60-250 | Econess Energy EN156P-60-250 | Econess Energy EN125M-96-255 | Econess Energy EN125M-96-260 | Econess Energy EN125M-96-265 | Econess Energy EN156M-72-280 | Econess Energy EN156P-72-280 | Econess Energy EN156M-72-285 | Econess Energy EN156P-72-285 | Econess Energy EN156M-72-290 | Econess Energy EN156P-72-290 | Econess Energy EN156M-72-295 | Econess Energy EN156P-72-295 | Econess Energy EN156M-72-300 | Econess Energy EN156P-72-300 | Ecosol PV Tech ECS195P-54 | Ecosol PV Tech ECS200P-54 | Ecosol PV Tech ECS205P-54 | Ecosol PV Tech ECS220P-60 | Ecosol PV Tech ECS225P-60 | Ecosol PV Tech ECS230P-60 | Ecosolargy TWES-(155)72M | Ecosolargy ECO160A125M-72 | Ecosolargy TWES-(160)72M | Ecosolargy ECO165A125M-72 | Ecosolargy SDM-170-(165)-72M | Ecosolargy TWES-(165)72M | Ecosolargy ECO170A125M-72 | Ecosolargy SDM-170-(170)-72M | Ecosolargy TWES-(170)72M | Ecosolargy ECO175A125M-72 | Ecosolargy SDM-170-(175)-72M | Ecosolargy TWES-(175)72M | Ecosolargy ECO180A125M-72 | Ecosolargy SDM-170-(180)-72M | Ecosolargy TWES-(180)72M | Ecosolargy ECO185A125M-72 | EcoSolargy ECO185S156P-54 | Ecosolargy SDM-170-(185)-72M | Ecosolargy ECO190A125M-72 | EcoSolargy ECO190S156P-54 | Ecosolargy ECO195A125M-72 | EcoSolargy ECO195S156P-54 | Ecosolargy ECO200A125M-72 | EcoSolargy ECO200S156P-54 | EcoSolargy ECO200S156P-60 | Ecosolargy TWES-(200)60P | EcoSolargy ECO205S156P-54 | EcoSolargy ECO205S156P-60 | Ecosolargy TWES-(205)60P | EcoSolargy ECO210S156P-54 | EcoSolargy ECO210S156P-60 | Ecosolargy TWES-(210)60P | EcoSolargy ECO215S156P-54 | EcoSolargy ECO215S156P-60 | Ecosolargy TWES-(215)60P | EcoSolargy ECO220S156P-54 | EcoSolargy ECO220S156P-60 | Ecosolargy TWES-(220)60P | EcoSolargy ECO225S156P-54 | EcoSolargy ECO225S156P-60 | Ecosolargy TWES-(225)60P | Ecosolargy ECO230A156M-60 | Ecosolargy ECO230A156P-60 | Ecosolargy ECO230A156PB-60 | Ecosolargy ECO230S156M-60 | EcoSolargy ECO230S156P-54 | EcoSolargy ECO230S156P-60 | Ecosolargy TWES-(230)60P | Ecosolargy ECO235A156M-60 | Ecosolargy ECO235A156P-60 | Ecosolargy ECO235A156PB-60 | EcoSolargy ECO235S156P-60 | Ecosolargy TWES-(235)60P | Ecosolargy ECO240A156M-60 | Ecosolargy ECO240A156P-60 | Ecosolargy ECO240A156PB-60 | Ecosolargy ECO240S156M-60 | EcoSolargy ECO240S156P-60 | EcoSolargy ECO240S156P-72 | Ecosolargy ECO245A156M-60 | Ecosolargy ECO245A156P-60 | EcoSolargy ECO245S156P-60 | EcoSolargy ECO245S156P-72 | Ecosolargy ECO250A156M-60 | Ecosolargy ECO250A156P-60 | Ecosolargy ECO250S156M-60 | EcoSolargy ECO250S156P-60 | EcoSolargy ECO250S156P-72 | EcoSolargy ECO255S156P-60 | EcoSolargy ECO255S156P-72 | EcoSolargy ECO260S156P-60 | EcoSolargy ECO260S156P-72 | EcoSolargy ECO265S156P-72 | EcoSolargy ECO270S156P-72 | Ecosolargy ECO275A156M-72 | Ecosolargy ECO275A156P-72 | EcoSolargy ECO275S156P-72 | Ecosolargy ECO280A156M-72 | Ecosolargy ECO280A156P-72 | EcoSolargy ECO280S156P-72 | Ecosolargy ECO285A156M-72 | Ecosolargy ECO285A156P-72 | EcoSolargy ECO285S156P-72 | Ecosolargy ECO290A156M-72 | Ecosolargy ECO290A156P-72 | EcoSolargy ECO290S156P-72 | Ecosolargy ECO295A156M-72 | Ecosolargy ECO295A156P-72 | EcoSolargy ECO295S156P-72 | Ecosolargy ECO300A156M-72 | EcoSolargy ECO300S156P-72 | ENN Solar Energy EST-110 | ENN Solar Energy EST-115A | ENN Solar Energy EST-115 | ENN Solar Energy EST-120 | ENN Solar Energy EST-220H | ENN Solar Energy EST-220V | ENN Solar Energy EST-228HA | ENN Solar Energy EST-228VA | ENN Solar Energy EST-230H | ENN Solar Energy EST-230V | ENN Solar Energy EST-240H | ENN Solar Energy EST-240V | ENN Solar Energy EST-440 | ENN Solar Energy EST-460 | ENN Solar Energy EST-460A | ENN Solar Energy EST-480 | Enp Sonne Solar Technikk ENP-M165MO | Enp Sonne Solar Technikk ENP-M170MO | Enp Sonne Solar Technikk ENP-M175MO | Enp Sonne Solar Technikk ENP-M180MO | Eoplly New Energy Technology EP125M-72-180W | Eoplly New Energy Technology EP125M-72-185W | Eoplly New Energy Technology EP125M-72-190W | Eoplly New Energy Technology EP125M-72-195W | Eoplly New Energy Technology EP125M-72-200W | Eoplly New Energy Technology EP125M-72-205W | Eoplly New Energy Technology EP125M-72-210W | Eoplly New Energy Technology EP156P-60-225S AC | Eoplly New Energy Technology EP156P-60-225W | Eoplly New Energy Technology EP156M-60-230S AC | Eoplly New Energy Technology EP156M-60-230W | Eoplly New Energy Technology EP156MB-60-230S AC | Eoplly New Energy Technology EP156MB-60-230W | Eoplly New Energy Technology EP156P-60-230S AC | Eoplly New Energy Technology EP156P-60-230W | Eoplly New Energy Technology EP156M-60-235S AC | Eoplly New Energy Technology EP156M-60-235W | Eoplly New Energy Technology EP156MB-60-235S AC | Eoplly New Energy Technology EP156MB-60-235W | Eoplly New Energy Technology EP156P-60-235S AC | Eoplly New Energy Technology EP156P-60-235W | Eoplly New Energy Technology EP156M-60-240S AC | Eoplly New Energy Technology EP156M-60-240W | Eoplly New Energy Technology EP156MB-60-240 AC | Eoplly New Energy Technology EP156MB-60-240S AC | Eoplly New Energy Technology EP156MB-60-240W | Eoplly New Energy Technology EP156P-60-240 AC | Eoplly New Energy Technology EP156P-60-240S AC | Eoplly New Energy Technology EP156P-60-240W | Eoplly New Energy Technology EP156M-60-245S AC | Eoplly New Energy Technology EP156M-60-245W | Eoplly New Energy Technology EP156MB-60-245 AC | Eoplly New Energy Technology EP156MB-60-245S AC | Eoplly New Energy Technology EP156MB-60-245W | Eoplly New Energy Technology EP156P-60-245 AC | Eoplly New Energy Technology EP156P-60-245S AC | Eoplly New Energy Technology EP156P-60-245W | Eoplly New Energy Technology EP156M-60-250 AC | Eoplly New Energy Technology EP156M-60-250S AC | Eoplly New Energy Technology EP156M-60-250W | Eoplly New Energy Technology EP156MB-60-250S AC | Eoplly New Energy Technology EP156MB-60-250W | Eoplly New Energy Technology EP156P-60-250S AC | Eoplly New Energy Technology EP156P-60-250W | Eoplly New Energy Technology EP156M-60-255 AC | Eoplly New Energy Technology EP156M-60-255S AC | Eoplly New Energy Technology EP156M-60-255W | Eoplly New Energy Technology EP156P-60-255S AC | Eoplly New Energy Technology EP156P-60-255W | Eoplly New Energy Technology EP156M-60-260 AC | Eoplly New Energy Technology EP156M-60-260S AC | Eoplly New Energy Technology EP156M-60-260W | Eoplly New Energy Technology EP156P-60-260S AC | Eoplly New Energy Technology EP156P-60-260W | Eoplly New Energy Technology EP156P-72-260W | Eoplly New Energy Technology EP156P-72-265W | Eoplly New Energy Technology EP156P-72-270W | Eoplly New Energy Technology EP156P-72-275W | Eoplly New Energy Technology EP156P-72-280W | Eoplly New Energy Technology EP156P-72-285W | Eoplly New Energy Technology EP156M-72-290W | Eoplly New Energy Technology EP156P-72-290W | Eoplly New Energy Technology EP156M-72-295W | Eoplly New Energy Technology EP156P-72-295W | Eoplly New Energy Technology EP156M-72-300W | Eoplly New Energy Technology EP156P-72-300W | Eoplly New Energy Technology EP156M-72-305W | Eoplly New Energy Technology EP156P-72-305W | Eoplly New Energy Technology EP156M-72-310W | Eoplly New Energy Technology EP156P-72-310W | Eoplly New Energy Technology EP156M-72-315W | Eoplly New Energy Technology EP156P-72-315W | Eoplly New Energy Technology EP156M-72-320W | Eoplly New Energy Technology EP156P-72-320W | ERA Solar ESPSA-170 | ERA Solar ESPSA-175 | ERA Solar ESPSA-180 | ERA Solar ESPSA-185 | ERA Solar ESPSA-190 | ERA Solar ESPSA-195 | ERA Solar ESPMC-205 | ERA Solar ESPMC-210 | ERA Solar ESPMC-215 | ERA Solar ESPMC-220 | ERA Solar ESPMC-225 | ERA Solar ESPMC-230 | ERA Solar ESPMC-235 | ERA Solar ESPMC-240 | ERA Solar ESPMC-245 | ET Solar Industry ET-M572165WW | ET Solar Industry ET-M572165WWZ | ET Solar Industry ET-M572170WW | ET Solar Industry ET-M572170WWZ | ET Solar Industry ET-M572175BB | ET Solar Industry ET-M572175BBZ | ET Solar Industry ET-M572175WW | ET Solar Industry ET-M572175WWZ | ET Solar Industry ET-M572180BB | ET Solar Industry ET-M572180BBZ | ET Solar Industry ET-M572180WW | ET Solar Industry ET-M572180WWZ | ET Solar Industry ET-M572185BB | ET Solar Industry ET-M572185BBZ | ET Solar Industry ET-M572185WW | ET Solar Industry ET-M572185WWZ | ET Solar Industry ET-M572190BBZ | ET Solar Industry ET-M572190WB | ET Solar Industry ET-M572190WW | ET Solar Industry ET-M572190WWZ | ET Solar Industry ET-P654190WB | ET Solar Industry ET-P654190WW | ET Solar Industry ET-P654195WB | ET Solar Industry ET-P654195WW | ET Solar Industry ET-P654200WB | ET Solar Industry ET-P654200WW | ET Solar Industry ET-P654205WB | ET Solar Industry ET-P654205WW | ET Solar Industry ET-P654210WB | ET Solar Industry ET-P654210WW | ET Solar Industry ET-P660220WB | ET Solar Industry ET-P660220WBZ | ET Solar Industry ET-P660220WW | ET Solar Industry ET-P660220WWZ | ET Solar Industry ET-A-P660225 | ET Solar Industry ET-A-P660225B | ET Solar Industry ET-P660225WB | ET Solar Industry ET-P660225WBZ | ET Solar Industry ET-P660225WW | ET Solar Industry ET-P660225WWZ | ET Solar Industry ET-A-P660230 | ET Solar Industry ET-A-P660230B | ET Solar Industry ET-P660230B | ET Solar Industry ET-P660230WB | ET Solar Industry ET-P660230WBZ | ET Solar Industry ET-P660230WW | ET Solar Industry ET-P660230WWZ | ET Solar Industry ET-A-M660235 | ET Solar Industry ET-A-M660235B | ET Solar Industry ET-A-P660235 | ET Solar Industry ET-A-P660235B | ET Solar Industry ET-P660235B | ET Solar Industry ET-P660235BB | ET Solar Industry ET-P660235BBZ | ET Solar Industry ET-P660235WB | ET Solar Industry ET-P660235WBZ | ET Solar Industry ET-P660235WW | ET Solar Industry ET-P660235WWZ | ET Solar Industry ET-A-M660240 | ET Solar Industry ET-A-M660240B | ET Solar Industry ET-A-P660240 | ET Solar Industry ET-A-P660240B | ET Solar Industry ET-P660240B | ET Solar Industry ET-P660240BB | ET Solar Industry ET-P660240BBZ | ET Solar Industry ET-P660240WB | ET Solar Industry ET-P660240WBZ | ET Solar Industry ET-P660240WW | ET Solar Industry ET-P660240WWZ | ET Solar Industry ET-A-M660245 | ET Solar Industry ET-A-M660245B | ET Solar Industry ET-A-P660245 | ET Solar Industry ET-A-P660245B | ET Solar Industry ET-P660245B | ET Solar Industry ET-P660245BAC | ET Solar Industry ET-P660245BB | ET Solar Industry ET-P660245BBAC | ET Solar Industry ET-P660245BBZ | ET Solar Industry ET-P660245BBZAC | ET Solar Industry ET-P660245WB | ET Solar Industry ET-P660245WBZ | ET Solar Industry ET-P660245WBZAC | ET Solar Industry ET-P660245WW | ET Solar Industry ET-P660245WWZ | ET Solar Industry ET-A-M660250 | ET Solar Industry ET-A-M660250B | ET Solar Industry ET-P660250BAC | ET Solar Industry ET-P660250BB | ET Solar Industry ET-P660250BBAC | ET Solar Industry ET-P660250BBZ | ET Solar Industry ET-P660250BBZAC | ET Solar Industry ET-P660250WB | ET Solar Industry ET-P660250WBZ | ET Solar Industry ET-P660250WBZAC | ET Solar Industry ET-P660250WW | ET Solar Industry ET-P660250WWZ | ET Solar Industry ET-P672250 | ET Solar Industry ET-A-M660255 | ET Solar Industry ET-A-M660255B | ET Solar Industry ET-P660255BB | ET Solar Industry ET-P660255BBZ | ET Solar Industry ET-P660255WB | ET Solar Industry ET-P660255WBZ | ET Solar Industry ET-P660255WW | ET Solar Industry ET-P660255WWZ | ET Solar Industry ET-P672255 | ET Solar Industry ET-A-M660260 | ET Solar Industry ET-A-M660260B | ET Solar Industry ET-P660260WB | ET Solar Industry ET-P660260WBZ | ET Solar Industry ET-P660260WW | ET Solar Industry ET-P660260WWZ | ET Solar Industry ET-P672260WB | ET Solar Industry ET-P672260WW | ET Solar Industry ET-A-M660265 | ET Solar Industry ET-A-M660265B | ET Solar Industry ET-P672265WB | ET Solar Industry ET-P672265WW | ET Solar Industry ET-P672270WB | ET Solar Industry ET-P672270WW | ET Solar Industry ET-A-P672275 | ET Solar Industry ET-A-P672275B | ET Solar Industry ET-P672275WB | ET Solar Industry ET-P672275WW | ET Solar Industry ET-A-P672280 | ET Solar Industry ET-A-P672280B | ET Solar Industry ET-P672280WB | ET Solar Industry ET-P672280WBG | ET Solar Industry ET-P672280WW | ET Solar Industry ET-P672280WWG | ET Solar Industry ET-A-M672285 | ET Solar Industry ET-A-M672285B | ET Solar Industry ET-A-P672285 | ET Solar Industry ET-A-P672285B | ET Solar Industry ET-P672285WB | ET Solar Industry ET-P672285WBG | ET Solar Industry ET-P672285WW | ET Solar Industry ET-P672285WWG | ET Solar Industry ET-A-M672290 | ET Solar Industry ET-A-M672290B | ET Solar Industry ET-A-P672290 | ET Solar Industry ET-A-P672290B | ET Solar Industry ET-P672290WB | ET Solar Industry ET-P672290WBG | ET Solar Industry ET-P672290WW | ET Solar Industry ET-P672290WWG | ET Solar Industry ET-A-M672295 | ET Solar Industry ET-A-M672295B | ET Solar Industry ET-A-P672295 | ET Solar Industry ET-A-P672295B | ET Solar Industry ET-P672295WB | ET Solar Industry ET-P672295WBG | ET Solar Industry ET-P672295WW | ET Solar Industry ET-P672295WWG | ET Solar Industry ET-A-M672300 | ET Solar Industry ET-A-M672300B | ET Solar Industry ET-P672300WB | ET Solar Industry ET-P672300WBG | ET Solar Industry ET-P672300WW | ET Solar Industry ET-P672300WWG | ET Solar Industry ET-A-M672305 | ET Solar Industry ET-A-M672305B | ET Solar Industry ET-P672305WB | ET Solar Industry ET-P672305WBG | ET Solar Industry ET-P672305WW | ET Solar Industry ET-P672305WWG | ET Solar Industry ET-P672310WB | ET Solar Industry ET-P672310WW | Exeltech AM24-1-B-6-0-00 | Exiom Solution EX-175M | Exiom Solution EX-175MB | Exiom Solution EX-180M | Exiom Solution EX-180MB | Exiom Solution EX-185M | Exiom Solution EX-185MB | Exiom Solution EX-185W | Exiom Solution EX-190M | Exiom Solution EX-195M | Exiom Solution EX-220P | Exiom Solution EX-220PB | Exiom Solution EX-225P | Exiom Solution EX-225PB | Exiom Solution EX-230P | Exiom Solution EX-230PB | Exiom Solution EX-230W | Exiom Solution EX-235P | Exiom Solution EX-235PB | Exiom Solution EX-235W | Exiom Solution EX-240P | Exiom Solution EX-240PB | Exiom Solution EX-240W | Exiom Solution EX-270P | Exiom Solution EX-270PB | Exiom Solution EX-275P | Exiom Solution EX-275PB | Exiom Solution EX-280P | Exiom Solution EX-280PB | Exiom Solution EX-285P | Exiom Solution EX-285PB | Exiom Solution EX-290P | Exiom Solution EX-290PB | Fire Energy FE5A-160M | Fire Energy FE6A-160P | Fire Energy FE6A-160PE | Fire Energy FE5A-170M | Fire Energy FE6A-170P | Fire Energy FE6P-170PE | Fire Energy FE5A-180M | Fire Energy FE6A-180P | Fire Energy FE6P-180PE | Fire Energy FE5A-190M | Fire Energy FE6P-190PE | Fire Energy FE6P-200PE | Fire Energy FE6P-210P | Fire Energy FE5P-220M | Fire Energy FE6P-220P | Fire Energy FE5P-230M | Fire Energy FE6P-230P | Fire Energy FE5P-240M | First Solar FS-267 | First Solar FS-367 | First Solar FS-270 | First Solar FS-370 | First Solar FS-272 | First Solar FS-372 | First Solar FS-275 | First Solar FS-375 | First Solar FS-277 | First Solar FS-377 | First Solar FS-280 | First Solar FS-380 | First Solar FS-382 | First Solar FS-385 | First Solar FS-387 | First Solar FS-390 | First Solar FS-392 | First Solar FS-395 | Fluitecnik FTS210P | Fluitecnik FTS215P | Fluitecnik FTS220P | Fluitecnik FTS225P | Fluitecnik FTS230M | Fluitecnik FTS230P | Fluitecnik FTS235M | Fluitecnik FTS240M | Fluitecnik FTS245M | Fluitecnik FTS250P | Fluitecnik FTS260P | Fluitecnik FTS270P | Fluitecnik FTS280P | Foxconn International FSM185-D4C0 | Foxconn International FSM190-D4C0 | Foxconn International FSM195-D4C0 | Foxconn International FSM205-D3C0 | Foxconn International FSM210-D3C0 | Foxconn International FSM215-D3C0 | Foxconn International FSM220-D3C0 | Foxconn International FSM225-D3C0 | Foxconn International FSM230-D2C0 | Foxconn International FSM235-D2C0 | Foxconn International FSM240-D2C0 | Foxconn International FSM245-D2C0 | Foxconn International FSM250-D2C0 | Foxconn International FSM275-D1E0 | Foxconn International FSM275-D1F0 | Foxconn International FSM280-D1E0 | Foxconn International FSM280-D1F0 | Foxconn International FSM285-D1E0 | Foxconn International FSM285-D1F0 | Foxconn International FSM290-D1E0 | Foxconn International FSM290-D1F0 | Foxconn International FSM295-D1E0 | Foxconn International FSM295-D1F0 | Future Solar Energy FSM572165 | Future Solar Energy FSM572170 | Future Solar Energy FSM572175 | Future Solar Energy FSM572180 | Future Solar Energy FSM572185 | Future Solar Energy FSP654195 | Future Solar Energy FSP654200 | Future Solar Energy FSP654205 | Future Solar Energy FSP654210 | Future Solar Energy FSP672260 | Future Solar Energy FSP672265 | Future Solar Energy FSP672270 | Future Solar Energy FSP672275 | Future Solar Energy FSP672280 | GCL-Poly (Suzhou) Energy GCL-P6-36-130 | GCL-Poly (Suzhou) Energy GCL-P6-36-135 | GCL-Poly (Suzhou) Energy GCL-P6-36-140 | GCL-Poly (Suzhou) Energy GCL-P6-36-145 | GCL-Poly (Suzhou) Energy GCL-P6-42-150 | GCL-Poly (Suzhou) Energy GCL-P6-42-155 | GCL-Poly (Suzhou) Energy GCL-P6-42-160 | GCL-Poly (Suzhou) Energy GCL-P6-42-165 | GCL-Poly (Suzhou) Energy GCL-P6-42-170 | GCL-Poly (Suzhou) Energy GCL-P6-48-170 | GCL-Poly (Suzhou) Energy GCL-P6-48-175 | GCL-Poly (SuZhou) Energy GCL-M5(L)-72-180 | GCL-Poly (Suzhou) Energy GCL-P6-48-180 | GCL-Poly (SuZhou) Energy GCL-M5(L)-72-185 | GCL-Poly (Suzhou) Energy GCL-P6-48-185 | GCL-Poly (SuZhou) Energy GCL-M5(L)-72-190 | GCL-Poly (Suzhou) Energy GCL-P6-48-190 | GCL-Poly (SuZhou) Energy GCL-M5(L)-72-195 | GCL-Poly (Suzhou) Energy GCL-P6-48-195 | GCL-Poly (SuZhou) Energy GCL-M5(L)-72-200 | GCL-Poly (Suzhou) Energy GCL-M6-60-200 | GCL-Poly (Suzhou) Energy GCL-P6-54-200 | GCL-Poly (SuZhou) Energy GCL-M5(L)-72-205 | GCL-Poly (Suzhou) Energy GCL-M6-60-205 | GCL-Poly (Suzhou) Energy GCL-P6-54-205 | GCL-Poly (SuZhou) Energy GCL-M5(L)-72-210 | GCL-Poly (Suzhou) Energy GCL-M6-60-210 | GCL-Poly (Suzhou) Energy GCL-P6-54-210 | GCL-Poly (Suzhou) Energy GCL-M6-60-215 | GCL-Poly (Suzhou) Energy GCL-P6-54-215 | GCL-Poly (Suzhou) Energy GCL-P6-60-215 | GCL-Poly (Suzhou) Energy GCL-M6-60-220 | GCL-Poly (Suzhou) Energy GCL-P6-54-220 | GCL-Poly (Suzhou) Energy GCL-P6-60-220 | GCL-Poly (Suzhou) Energy GCL-M6-60-225 | GCL-Poly (Suzhou) Energy GCL-P6-60-225 | GCL-Poly (Suzhou) Energy GCL-M6-60-230 | GCL-Poly (Suzhou) Energy GCL-P6-60-230 | GCL-Poly (Suzhou) Energy GCL-M6-60-235 | GCL-Poly (Suzhou) Energy GCL-P6-60-235 | GCL-Poly (Suzhou) Energy GCL-M6-60-240 | GCL-Poly (Suzhou) Energy GCL-P6-60-240 | GCL-Poly (Suzhou) Energy GCL-P6-60-245 | GCL-Poly (Suzhou) Energy GCL-P6-60-250 | GCL-Poly (Suzhou) Energy GCL-P6-72-250 | GCL-Poly (Suzhou) Energy GCL-P6-72-255 | GCL-Poly (Suzhou) Energy GCL-P6-72-260 | GCL-Poly (Suzhou) Energy GCL-P6-72-265 | GCL-Poly (Suzhou) Energy GCL-P6-72-270 | GCL-Poly (Suzhou) Energy GCL-P6-72-275 | GCL-Poly (Suzhou) Energy GCL-P6-72-280 | GCL-Poly (Suzhou) Energy GCL-P6-72-285 | GCL-Poly (Suzhou) Energy GCL-P6-72-290 | GCL-Poly (Suzhou) Energy GCL-P6-72-295 | GCL-Poly (Suzhou) Energy GCL-P6-72-300 | GCL-Poly (Suzhou) Energy GCL-P6-72-305 | GCL-Poly (Suzhou) Energy GCL-P6-72-310 | GCL-Poly (Suzhou) Energy GCL-P6-72-315 | GCL-Poly (Suzhou) New Energy Limited GCL-P6-36-130 | GCL-Poly (Suzhou) New Energy Limited GCL-P6-36-135 | GCL-Poly (Suzhou) New Energy Limited GCL-P6-36-140 | GCL-Poly (Suzhou) New Energy Limited GCL-P6-36-145 | GCL-Poly (Suzhou) New Energy Limited GCL-P6-42-150 | GCL-Poly (Suzhou) New Energy Limited GCL-P6-42-155 | GCL-Poly (Suzhou) New Energy Limited GCL-P6-42-160 | GCL-Poly (Suzhou) New Energy Limited GCL-P6-42-165 | GCL-Poly (Suzhou) New Energy Limited GCL-P6-42-170 | GCL-Poly (Suzhou) New Energy Limited GCL-P6-48-170 | GCL-Poly (Suzhou) New Energy Limited GCL-P6-48-175 | GCL-Poly (Suzhou) New Energy Limited GCL-P6-48-180 | GCL-Poly (Suzhou) New Energy Limited GCL-P6-48-185 | GCL-Poly (Suzhou) New Energy Limited GCL-P6-48-190 | GCL-Poly (Suzhou) New Energy Limited GCL-P6-48-195 | GCL-Poly (Suzhou) New Energy Limited GCL-P6-54-200 | GCL-Poly (Suzhou) New Energy Limited GCL-P6-54-205 | GCL-Poly (Suzhou) New Energy Limited GCL-P6-54-210 | GCL-Poly (Suzhou) New Energy Limited GCL-P6-54-215 | GCL-Poly (Suzhou) New Energy Limited GCL-P6-54-220 | GCL-Poly (Suzhou) New Energy Limited GCL-P6-60-220 | GCL-Poly (Suzhou) New Energy Limited GCL-P6-60-225 | GCL-Poly (Suzhou) New Energy Limited GCL-P6-60-230 | GCL-Poly (Suzhou) New Energy Limited GCL-P6-60-235 | GCL-Poly (Suzhou) New Energy Limited GCL-P6-60-240 | General Energy Solutions 7C00-6A225 | General Energy Solutions 7C00-6A230 | General Energy Solutions 7C00-6A235 | General Energy Solutions 7E00-6A235 | General Energy Solutions 7C00-6A240 | General Energy Solutions 7E00-6A240 | General Energy Solutions 7C00-6A245 | General Energy Solutions 7E00-6A245 | General Energy Solutions 7E00-6A250 | General Energy Solutions 7E00-6A255 | General Energy Solutions 7E00-6A260 | General Energy Solutions 7E00-6A265 | General Energy Solutions 7C00-6C275 | General Energy Solutions 7C00-6C280 | General Energy Solutions 7C00-6C285 | General Energy Solutions 7E00-6C285 | General Energy Solutions 7C00-6C290 | General Energy Solutions 7E00-6C290 | General Energy Solutions 7C00-6C295 | General Energy Solutions 7E00-6C295 | General Energy Solutions 7C00-6C300 | General Energy Solutions 7E00-6C300 | General Energy Solutions 7C00-6C305 | General Energy Solutions 7E00-6C305 | General Energy Solutions 7C00-6C310 | General Energy Solutions 7E00-6C310 | General Energy Solutions 7E00-6C315 | General Solar Power (Yantai) GSC90UR33Y | General Solar Power (Yantai) GSC93UR33Y | General Solar Power (Yantai) GSB94UR33 | General Solar Power (Yantai) GSB97UR33 | General Solar Power (Yantai) GSB100UR33 | GESOLAR GES-M165 | GESOLAR GES-M170 | GESOLAR GES-M175 | GESOLAR GES-M180 | GESOLAR GES-P200 | GESOLAR GES-P210 | GESOLAR GES-P220 | GESOLAR GES-P230 | GESOLAR GES-P240 | GESOLAR GES-P250 | GESOLAR GES-P260 | GESOLAR GES-P270 | GESOLAR GES-P280 | Gintech Energy GTE 200M | Gintech Energy GTE 205M | Gintech Energy GTE 210M | Gintech Energy GTE 215M | Gintech Energy GTE 220M | Gintech Energy GTE 225M | Gintech Energy GTE 230M | Gintech Energy GTE 235M | Gintech Energy GTE 240M | Global Solar Energy FG-2BTM-82 | Global Solar Energy FG-2BTN-82 | Global Solar Energy FG-2BTM-90 | Global Solar Energy FG-2BTN-90 | Global Solar Energy FG-2BTM-100 | Global Solar Energy FG-2BTN-100 | Global Solar Energy FG-1BTM-225 | Global Solar Energy FG-1BTN-225 | Global Solar Energy FG-1BTM-250 | Global Solar Energy FG-1BTN-250 | Global Solar Energy FG-1BTM-275 | Global Solar Energy FG-1BTN-275 | Global Solar Energy FG-1BTM-300 | Global Solar Energy FG-1BTN-300 | Global Sun P-220GS | Global Sun P-225GS | Global Sun P-230GS | Global Sun P-235GS | Global Sun P-240GS | Gloria Solar GSS5-160A-E1 | Gloria Solar GSS5-165A-E1 | Gloria Solar GSS5-170A-E1 | Gloria Solar GSS5-175A-E1 | Gloria Solar GSS5-180A-E1 | Gloria Solar GSM6-200D-E1 | Gloria Solar GSM6-205D-E1 | Gloria Solar GSM6-210D-E1 | Gloria Solar GSM6-215D-E1 | Gloria Solar GSM6-220D-E1 | Gloria Solar GSM6-225D-E1 | Gloria Solar GSM6-230D-E1 | Gloria Solar GSM6-235D-E1 | Gloria Solar GSM6-240D-E1 | Grape Solar GS-P-120-PDX | Grape Solar GS-P-125-PDX | Grape Solar GS-P-130-PDX | Grape Solar GS-P-135-PDX | Grape Solar GS-P-140-PDX | Grape Solar GS-S-150-SF | Grape Solar GS-S-155-SF | Grape Solar GS-P-160-EUG | Grape Solar GS-S-160-Fab8 | Grape Solar GS-S-160-SF | Grape Solar CS-S-165-DJ | Grape Solar GS-P-165-EUG | Grape Solar GS-S-165-Fab8 | Grape Solar GS-S-165-SF | Grape Solar CS-S-170-DJ | Grape Solar GS-P-170-EUG | Grape Solar GS-S-170-Fab3 | Grape Solar GS-S-170-SF | Grape Solar GS-S-175-Fab8 | Grape Solar CS-S-175-DJ | Grape Solar GS-P-175-EUG | Grape Solar GS-S-175-EUG | Grape Solar GS-S-175-Fab3 | Grape Solar GS-S-175-SF | Grape Solar CS-S-180-DJ | Grape Solar GS-P-180-EUG | Grape Solar GS-S-180-EUG | Grape Solar GS-S-180-Fab3 | Grape Solar GS-S-180-Fab8 | Grape Solar GS-S-180-SF | Grape Solar GS-S-185-Fab3 | Grape Solar GS-S-185-Fab8 | Grape Solar GS-S-185-SF | Grape Solar GS-P-190-EUG | Grape Solar GS-S-190-Fab3 | Grape Solar GS-P-190-SL6-18 | Grape Solar GS-P-195-EUG | Grape Solar GS-S-195-Fab3 | Grape Solar CS-P-200-DJ | Grape Solar GS-P-200-CSPE | Grape Solar GS-P-200-EUG | Grape Solar GS-P-200-Fab1 | Grape Solar GS-P-200-OR | Grape Solar GS-P-200-PDX | Grape Solar GS-P-200-SL6-18 | Grape Solar GS-S-200-Fab1 | Grape Solar GS-P-205-EUG | Grape Solar GS-P-205-Fab1 | Grape Solar GS-P-205-OR | Grape Solar GS-P-205-PDX | Grape Solar GS-P-205-SL6-18 | Grape Solar GS-S-205-Fab1 | Grape Solar CS-P-210-DJ | Grape Solar GS-P-210-Fab1 | Grape Solar GS-P-210-Fab5 | Grape Solar GS-P-210-OR | Grape Solar GS-P-210-PDX | Grape Solar GS-S-210-Fab1 | Grape Solar GS-P-215-Fab1 | Grape Solar GS-P-215-Fab5 | Grape Solar GS-P-215-OR | Grape Solar GS-P-215-PDX | Grape Solar GS-S-215-Fab1 | Grape Solar CS-P-220-DJ | Grape Solar GS-P-220-CS | Grape Solar GS-P-220-EUG | Grape Solar GS-P-220-Fab1 | Grape Solar GS-P-220-Fab5 | Grape Solar GS-P-220-OR | Grape Solar GS-P-220-PDX | Grape Solar GS-P-220-SL6-20 | Grape Solar GS-S-220-CS | Grape Solar GS-S-220-Fab1 | Grape Solar GS-S-220-Fab3 | Grape Solar GS-S-220-Fab8 | Grape Solar GS-P-225-EUG | Grape Solar GS-P-225-Fab1 | Grape Solar GS-P-225-Fab5 | Grape Solar GS-P-225-PDX | Grape Solar GS-P-225-SL6-20 | Grape Solar GS-S-225-Fab1 | Grape Solar GS-S-225-Fab3 | Grape Solar GS-S-225-Fab8 | Grape Solar CS-P-230-DJ | Grape Solar GS-P-230-CS | Grape Solar GS-P-230-EUG | Grape Solar GS-P-230-Fab1 | Grape Solar GS-P-230-Fab5 | Grape Solar GS-P-230-PDX | Grape Solar GS-P-230-SL6-20 | Grape Solar GS-S-230-CS | Grape Solar GS-S-230-Fab1 | Grape Solar GS-S-230-Fab3 | Grape Solar GS-S-230-Fab8 | Grape Solar GS-P-235-Fab1 | Grape Solar GS-P-235-Fab5 | Grape Solar GS-P-235-PDX | Grape Solar GS-S-235-Fab1 | Grape Solar GS-S-235-Fab3 | Grape Solar GS-S-235-Fab8 | Grape Solar CS-P-240-DJ | Grape Solar GS-P-240-Fab1 | Grape Solar GS-P-240-PDX | Grape Solar GS-S-240-CS | Grape Solar GS-S-240-Fab1 | Grape Solar GS-S-240-Fab3 | Grape Solar GS-S-240-Fab8 | Grape Solar GS-P-245-PDX | Grape Solar GS-S-245-Fab3 | Grape Solar GS-S-245-Fab8 | Grape Solar CS-P-250-DJ | Grape Solar GS-P-250-EUG | Grape Solar GS-P-250-PDX | Grape Solar GS-S-250-Fab3 | Grape Solar GS-S-250-Fab5 | Grape Solar GS-S-250-Fab8 | Grape Solar GS-P-255-EUG | Grape Solar GS-P-255-PDX | Grape Solar GS-S-255-Fab3 | Grape Solar GS-S-255-Fab5 | Grape Solar CS-P-260-DJ | Grape Solar GS-P-260-EUG | Grape Solar GS-P-260-Fab1 | Grape Solar GS-P-260-PDX | Grape Solar GS-S-260-Fab1 | Grape Solar GS-S-260-Fab5 | Grape Solar GS-P-265-Fab1 | Grape Solar GS-P-265-PDX | Grape Solar GS-S-265-Fab1 | Grape Solar GS-S-265-Fab5 | Grape Solar CS-P-270-DJ | Grape Solar GS-P-270-EUG | Grape Solar GS-P-270-Fab1 | Grape Solar GS-P-270-PDX | Grape Solar GS-S-270-Fab1 | Grape Solar GS-S-270-Fab5 | Grape Solar GS-P-275-EUG | Grape Solar GS-P-275-Fab1 | Grape Solar GS-P-275-PDX | Grape Solar GS-S-275-Fab1 | Grape Solar GS-S-275-Fab5 | Grape Solar CS-P-280-DJ | Grape Solar GS-P-280-EUG | Grape Solar GS-P-280-Fab1 | Grape Solar GS-P-280-PDX | Grape Solar GS-S-280-Fab1 | Grape Solar GS-S-280-Fab5 | Grape Solar GS-P-285-Fab1 | Grape Solar GS-P-285-FAB36 | Grape Solar GS-P-285-PDX | Grape Solar GS-S-285-Fab1 | Grape Solar GS-P-290-Fab1 | Grape Solar GS-P-290-FAB36 | Grape Solar GS-S-290-Fab1 | Grape Solar GS-S-290-FAB36 | Grape Solar GS-P-295-Fab1 | Grape Solar GS-P-295-FAB36 | Grape Solar GS-S-295-Fab1 | Grape Solar GS-S-295-FAB36 | Grape Solar GS-P-300-FAB36 | Grape Solar GS-S-300-FAB36 | Grape Solar GS-S-305-FAB36 | Grape Solar GS-S-310-FAB36 | Grape Solar GS-S-385-TS | Grape Solar GS-S-390-TS | Grape Solar GS-S-395-Platinum | Grape Solar GS-S-400-Platinum | Grape Solar GS-S-405-Platinum | Grape Solar GS-S-410-Platinum | Green Energy Solar & Wind GESW1750 USA-170W | Green Energy Solar & Wind GESW1750 USA-175W | Green Energy Solar & Wind GESW1750 USA-180W | Green Energy Solar & Wind GESW2100 USA-210W | Green Energy Solar & Wind GESW2100 USA-215W | Green Energy Solar & Wind GESW2100 USA-220W | Green Energy Technology GET-085A | Green Energy Technology GET-090A | Green Energy Technology GET-095A-1 | Green Energy Technology GET-095-AT | Green Energy Technology GET-100A-1 | Green Energy Technology GET-100-AT | Green Energy Technology GET-105-AT | Green Energy Technology GET-170A | Green Energy Technology GET-170B | Green Energy Technology GET-180A | Green Energy Technology GET-180B | Green Energy Technology GET-340A | Green Energy Technology GET-360A | Green Power ET-M572165 | Green Power ET-M572170 | Green Power ET-M572175 | Green Power ET-M572175B | Green Power ET-M572180 | Green Power ET-M572180B | Green Power ET-M572185 | Green Power ET-M572185B | Green Power ET-P654190B | Green Power ET-P654195 | Green Power ET-P654195B | Green Power ET-P654200 | Green Power ET-P654200B | Green Power ET-P654205 | Green Power ET-P654205B | Green Power ET-P654210 | Green Power ET-P654210B | Green Power ET-P660220 | Green Power ET-P660220B | Green Power ET-P660225 | Green Power ET-P660225B | Green Power ET-P660230 | Green Power ET-P660230B | Green Power ET-P660235 | Green Power ET-P660235B | Green Power ET-P672260 | Green Power ET-P672260B | Green Power ET-P672265 | Green Power ET-P672265B | Green Power ET-P672270 | Green Power ET-P672270B | Green Power ET-P672275 | Green Power ET-P672275B | Green Power ET-P672280 | Green Power ET-P672280B | Greenbrilliance Energy GB54P6-200 | Greenbrilliance Energy GB60P6-210 | Greenbrilliance Energy GB60P6-215 | Greenbrilliance Energy GB60P6-220 | Greenbrilliance Energy GB60P6-225 | Greenbrilliance Energy GB60P6-230 | Greenbrilliance Energy GB72P6-270 | Greenbrilliance Energy GB72P6-275 | Greenbrilliance Energy GB72P6-280 | Greenlite Solar Canada GLS-200 | Greenlite Solar Canada GLS-220 | Greenlite Solar Canada GLS-270 | GS-Solar (Fujian) GS-46SU | GS-Solar (Fujian) GS-58 | GS-Solar (Fujian) GS-60 | GS-Solar (Fujian) GS-63 | Guangdong Fivestar Solar Energy FS-M125-175W | Guangdong Fivestar Solar Energy FS-P156-210W | Guangdong Fivestar Solar Energy FS-P156-220W | Guangdong Golden Glass Technologies GG160M2-24-1324x992 | Guangdong Golden Glass Technologies GG165M2-24-1324x992 | Guangdong Golden Glass Technologies GG170M2-24-1324x992 | Guangdong Golden Glass Technologies GG175M2-24-1324x992 | Guangdong Golden Glass Technologies GG175S1-36-1589x807 | Guangdong Golden Glass Technologies GG180M2-24-1324x992 | Guangdong Golden Glass Technologies GG180S1-36-1589x807 | Guangdong Golden Glass Technologies GG190M2-27-1482x992 | Guangdong Golden Glass Technologies GG195M2-27-1482x992 | Guangdong Golden Glass Technologies GG200M2-27-1482x992 | Guangdong Golden Glass Technologies GG205M2-27-1482x992 | Guangdong Golden Glass Technologies GG220M2-30-1640x992 | Guangdong Golden Glass Technologies GG225M2-30-1640x992 | Guangdong Golden Glass Technologies GG230M2-30-1640x992 | Guangdong Golden Glass Technologies GG250M2-35-1956x992 | Guangdong Golden Glass Technologies GG255M2-35-1956x992 | Guangdong Golden Glass Technologies GG260M2-35-1956x992 | Guangdong Golden Glass Technologies GG270M2-36-1956x992 | Guangdong Golden Glass Technologies GG275M2-36-1956x992 | Guangdong Golden Glass Technologies GG280M2-36-1956x992 | Guodian Jintech Solar Energy JT5M-175-E | Guodian Jintech Solar Energy JT5M-180-E | Guodian Jintech Solar Energy JT5M-185-E | Guodian Jintech Solar Energy JT6P-215-D | Guodian Jintech Solar Energy JT6P-220-D | Guodian Jintech Solar Energy JT6P-225-D | Guodian Jintech Solar Energy JT6P-230-D | Guodian Jintech Solar Energy JT6P-235-D | Guodian Jintech Solar Energy JT6P-255-E | Guodian Jintech Solar Energy JT6P-260-E | Guodian Jintech Solar Energy JT6P-265-E | Guodian Jintech Solar Energy JT6P-270-E | Guodian Jintech Solar Energy JT6P-275-E | Guodian Jintech Solar Energy JT6P-280-E | Hangzhou AmpleSun Solar Technology ASF100 | Hangzhou Zhejiang University Sunny Energy Science&Tech ZDNY-180C | Hangzhou Zhejiang University Sunny Energy Science&Tech ZDNY-185C | Hangzhou Zhejiang University Sunny Energy Science&Tech ZDNY-190C | Hangzhou Zhejiang University Sunny Energy Science&Tech ZDNY-200P54 | Hangzhou Zhejiang University Sunny Energy Science&Tech ZDNY-210C54 | Hangzhou Zhejiang University Sunny Energy Science&Tech ZDNY-210P54 | Hangzhou Zhejiang University Sunny Energy Science&Tech ZDNY-220C54 | Hangzhou Zhejiang University Sunny Energy Science&Tech ZDNY-220P54 | Hangzhou Zhejiang University Sunny Energy Science&Tech ZDNY-220P60 | Hangzhou Zhejiang University Sunny Energy Science&Tech ZDNY-230C54 | Hangzhou Zhejiang University Sunny Energy Science&Tech ZDNY-230C60 | Hangzhou Zhejiang University Sunny Energy Science&Tech ZDNY-230P60 | Hangzhou Zhejiang University Sunny Energy Science&Tech ZDNY-240C60 | Hangzhou Zhejiang University Sunny Energy Science&Tech ZDNY-240P60 | Hangzhou Zhejiang University Sunny Energy Science&Tech ZDNY-250C60 | Hangzhou Zhejiang University Sunny Energy Science&Tech ZDNY-270P72 | Hangzhou Zhejiang University Sunny Energy Science&Tech ZDNY-280C72 | Hangzhou Zhejiang University Sunny Energy Science&Tech ZDNY-280P72 | Hangzhou Zhejiang University Sunny Energy Science&Tech ZDNY-290C72 | Hangzhou Zhejiang University Sunny Energy Science&Tech ZDNY-290P72 | Hangzhou Zhejiang University Sunny Energy Science&Tech ZDNY-300C72 | Hansol Technics HS238SB-A | Hansol Technics HS238SB-A06 | Hansol Technics HS240SB-A | Hansol Technics HS240SB-A06 | Hansol Technics HS243SB-A | Hansol Technics HS243SB-A06 | Hansol Technics HS245SB-A | Hansol Technics HS245SB-A06 | Hansol Technics HS248SB-A | Hansol Technics HS248SB-A06 | Hansol Technics HS250SB-A | Hansol Technics HS250SB-A06 | Hansol Technics HS253SB-A | Hansol Technics HS253SB-A06 | Hansol Technics HS255SB-A | Hansol Technics HS255SB-A06 | Hansol Technics HS258SB-A | Hansol Technics HS258SB-A06 | Hansol Technics HS260SB-A | Hansol Technics HS260SB-A06 | Hanwha Q-Cells Q.PRO L 290 | Hanwha Q-Cells Q.PRO L 295 | Hanwha Q-Cells Q.PRO L 300 | Hanwha Q-Cells Q.PRO L 305 | Hanwha SolarOne (Qidong) SF160-24-M150 | Hanwha SolarOne (Qidong) SF160-24-M155 | Hanwha SolarOne (Qidong) SF160-24-M160 | Hanwha SolarOne (Qidong) SF160-24-M160B | Hanwha SolarOne (Qidong) SF160-24-M165 | Hanwha SolarOne (Qidong) SF160-24-M165B | Hanwha SolarOne (Qidong) SF160-24-P165 | Hanwha SolarOne (Qidong) SF160-24-M170 | Hanwha SolarOne (Qidong) SF160-24-M170B | Hanwha SolarOne (Qidong) SF160-24-P170 | Hanwha SolarOne (Qidong) SF190-27-P170 | Hanwha SolarOne (Qidong) SF160-24-M175 | Hanwha SolarOne (Qidong) SF160-24-M175B | Hanwha SolarOne (Qidong) SF160-24-M175L | Hanwha SolarOne (Qidong) SF160-24-M175L-B | Hanwha SolarOne (Qidong) SF160-24-P175 | Hanwha SolarOne (Qidong) SF190-27-P175 | Hanwha SolarOne (Qidong) SF160-24-M180 | Hanwha SolarOne (Qidong) SF160-24-M180B | Hanwha SolarOne (Qidong) SF160-24-M180L | Hanwha SolarOne (Qidong) SF160-24-M180L-B | Hanwha SolarOne (Qidong) SF190-27-M180 | Hanwha SolarOne (Qidong) SF190-27-M180B | Hanwha SolarOne (Qidong) SF190-27-P180 | Hanwha SolarOne (Qidong) SF160-24-M185 | Hanwha SolarOne (Qidong) SF160-24-M185B | Hanwha SolarOne (Qidong) SF160-24-M185L | Hanwha SolarOne (Qidong) SF160-24-M185L-B | Hanwha SolarOne (Qidong) SF190-27-M185 | Hanwha SolarOne (Qidong) SF190-27-M185B | Hanwha SolarOne (Qidong) SF190-27-P185 | Hanwha SolarOne (Qidong) SF160-24-M190 | Hanwha SolarOne (Qidong) SF160-24-M190B | Hanwha SolarOne (Qidong) SF160-24-M190L | Hanwha SolarOne (Qidong) SF160-24-M190L-B | Hanwha SolarOne (Qidong) SF190-27-M190 | Hanwha SolarOne (Qidong) SF190-27-M190B | Hanwha SolarOne (Qidong) SF190-27-P190 | Hanwha SolarOne (Qidong) SF190-27-M195 | Hanwha SolarOne (Qidong) SF190-27-M195B | Hanwha SolarOne (Qidong) SF190-27-P195 | Hanwha SolarOne (Qidong) SF190-27-M200 | Hanwha SolarOne (Qidong) SF190-27-M200B | Hanwha SolarOne (Qidong) SF190-27-P200 | Hanwha SolarOne (Qidong) SF220-30-M200 | Hanwha SolarOne (Qidong) SF220-30-M200B | Hanwha SolarOne (Qidong) SF220-30-P200 | Hanwha SolarOne (Qidong) SF220-30-P200B | Hanwha SolarOne (Qidong) SF190-27-M205 | Hanwha SolarOne (Qidong) SF190-27-M205B | Hanwha SolarOne (Qidong) SF190-27-P205 | Hanwha SolarOne (Qidong) SF220-30-M205 | Hanwha SolarOne (Qidong) SF220-30-M205B | Hanwha SolarOne (Qidong) SF220-30-P205 | Hanwha SolarOne (Qidong) SF220-30-P205B | Hanwha SolarOne (Qidong) SF190-27-M210 | Hanwha SolarOne (Qidong) SF190-27-M210B | Hanwha SolarOne (Qidong) SF190-27-P210 | Hanwha SolarOne (Qidong) SF220-30-M210 | Hanwha SolarOne (Qidong) SF220-30-M210B | Hanwha SolarOne (Qidong) SF220-30-P210 | Hanwha SolarOne (Qidong) SF220-30-P210B | Hanwha SolarOne (Qidong) SF220-30-M215 | Hanwha SolarOne (Qidong) SF220-30-M215B | Hanwha SolarOne (Qidong) SF220-30-P215 | Hanwha SolarOne (Qidong) SF220-30-P215B | Hanwha SolarOne (Qidong) SF220-30-M220 | Hanwha SolarOne (Qidong) SF220-30-M220B | Hanwha SolarOne (Qidong) SF220-30-P220 | Hanwha SolarOne (Qidong) SF220-30-P220B | Hanwha SolarOne (Qidong) SF220-30-M225 | Hanwha SolarOne (Qidong) SF220-30-M225B | Hanwha SolarOne (Qidong) SF220-30-P225 | Hanwha SolarOne (Qidong) SF220-30-P225B | Hanwha SolarOne (Qidong) HSL60P6-PA-3-230Q | Hanwha SolarOne (Qidong) HSL60P6-PA-3-230QB | Hanwha SolarOne (Qidong) HSL60P6-PA-3-230QW | Hanwha SolarOne (Qidong) HSL60P6-PB-3-230Q | Hanwha SolarOne (Qidong) HSL60P6-PB-3-230QB | Hanwha SolarOne (Qidong) HSL60P6-PB-3-230QW | Hanwha SolarOne (Qidong) SF220-30-M230 | Hanwha SolarOne (Qidong) SF220-30-M230B | Hanwha SolarOne (Qidong) SF220-30-M230L | Hanwha SolarOne (Qidong) SF220-30-P230 | Hanwha SolarOne (Qidong) SF220-30-P230B | Hanwha SolarOne (Qidong) SF220-30-P230L | Hanwha SolarOne (Qidong) SF220-30-P230L-B | Hanwha Solarone (Qidong) HSL60P6-PA-0-235T | Hanwha SolarOne (Qidong) HSL60P6-PA-0-235TB | Hanwha SolarOne (Qidong) HSL60P6-PA-0-235TW | Hanwha SolarOne (Qidong) HSL60P6-PA-2-235Q | Hanwha SolarOne (Qidong) HSL60P6-PA-2-235QB | Hanwha SolarOne (Qidong) HSL60P6-PA-2-235QW | Hanwha SolarOne (Qidong) HSL60P6-PA-3-235Q | Hanwha SolarOne (Qidong) HSL60P6-PA-3-235QB | Hanwha SolarOne (Qidong) HSL60P6-PA-3-235QW | Hanwha SolarOne (Qidong) HSL60P6-PA-4-235Q | Hanwha SolarOne (Qidong) HSL60P6-PA-4-235QB | Hanwha SolarOne (Qidong) HSL60P6-PA-4-235QW | Hanwha SolarOne (Qidong) HSL60P6-PA-4-235T | Hanwha SolarOne (Qidong) HSL60P6-PA-4-235TB | Hanwha SolarOne (Qidong) HSL60P6-PA-4-235TW | Hanwha SolarOne (Qidong) HSL60P6-PB-2-235Q | Hanwha SolarOne (Qidong) HSL60P6-PB-2-235QB | Hanwha SolarOne (Qidong) HSL60P6-PB-2-235QW | Hanwha SolarOne (Qidong) HSL60P6-PB-3-235Q | Hanwha SolarOne (Qidong) HSL60P6-PB-3-235QB | Hanwha SolarOne (Qidong) HSL60P6-PB-3-235QW | Hanwha SolarOne (Qidong) HSL60P6-PB-4-235Q | Hanwha SolarOne (Qidong) HSL60P6-PB-4-235QB | Hanwha SolarOne (Qidong) HSL60P6-PB-4-235QW | Hanwha SolarOne (Qidong) SF220-30-M235 | Hanwha SolarOne (Qidong) SF220-30-M235B | Hanwha SolarOne (Qidong) SF220-30-M235L | Hanwha SolarOne (Qidong) SF220-30-P235 | Hanwha SolarOne (Qidong) SF220-30-P235B | Hanwha SolarOne (Qidong) SF220-30-P235L | Hanwha SolarOne (Qidong) SF220-30-P235L-B | Hanwha SolarOne (Qidong) HSL60M6-HA-0-240T | Hanwha SolarOne (Qidong) HSL60M6-HA-0-240TW | Hanwha SolarOne (Qidong) HSL60M6-HA-4-240T | Hanwha SolarOne (Qidong) HSL60M6-HA-4-240TB | Hanwha SolarOne (Qidong) HSL60M6-HA-4-240TW | Hanwha SolarOne (Qidong) HSL60M6-HB-0-240T | Hanwha SolarOne (Qidong) HSL60M6-HB-0-240TB | Hanwha SolarOne (Qidong) HSL60M6-HB-0-240TW | Hanwha SolarOne (Qidong) HSL60M6-HB-4-240T | Hanwha SolarOne (Qidong) HSL60M6-HB-4-240TB | Hanwha SolarOne (Qidong) HSL60M6-HB-4-240TW | Hanwha Solarone (Qidong) HSL60P6-PA-0-240T | Hanwha SolarOne (Qidong) HSL60P6-PA-0-240TB | Hanwha SolarOne (Qidong) HSL60P6-PA-0-240TW | Hanwha SolarOne (Qidong) HSL60P6-PA-2-240Q | Hanwha SolarOne (Qidong) HSL60P6-PA-2-240QB | Hanwha SolarOne (Qidong) HSL60P6-PA-2-240QW | Hanwha SolarOne (Qidong) HSL60P6-PA-3-240Q | Hanwha SolarOne (Qidong) HSL60P6-PA-3-240QB | Hanwha SolarOne (Qidong) HSL60P6-PA-3-240QW | Hanwha SolarOne (Qidong) HSL60P6-PA-4-240Q | Hanwha SolarOne (Qidong) HSL60P6-PA-4-240QB | Hanwha SolarOne (Qidong) HSL60P6-PA-4-240QW | Hanwha SolarOne (Qidong) HSL60P6-PA-4-240T | Hanwha SolarOne (Qidong) HSL60P6-PA-4-240TB | Hanwha SolarOne (Qidong) HSL60P6-PA-4-240TW | Hanwha Solarone (Qidong) HSL60P6-PB-0-240T | Hanwha SolarOne (Qidong) HSL60P6-PB-0-240TB | Hanwha SolarOne (Qidong) HSL60P6-PB-0-240TW | Hanwha SolarOne (Qidong) HSL60P6-PB-2-240Q | Hanwha SolarOne (Qidong) HSL60P6-PB-2-240QB | Hanwha SolarOne (Qidong) HSL60P6-PB-2-240QW | Hanwha SolarOne (Qidong) HSL60P6-PB-3-240Q | Hanwha SolarOne (Qidong) HSL60P6-PB-3-240QB | Hanwha SolarOne (Qidong) HSL60P6-PB-3-240QW | Hanwha SolarOne (Qidong) HSL60P6-PB-4-240Q | Hanwha SolarOne (Qidong) HSL60P6-PB-4-240QB | Hanwha SolarOne (Qidong) HSL60P6-PB-4-240QW | Hanwha SolarOne (Qidong) HSL60P6-PB-4-240T | Hanwha SolarOne (Qidong) HSL60P6-PB-4-240TB | Hanwha SolarOne (Qidong) HSL60P6-PB-4-240TW | Hanwha SolarOne (Qidong) SF220-30-M240 | Hanwha SolarOne (Qidong) SF220-30-M240B | Hanwha SolarOne (Qidong) SF220-30-M240L | Hanwha SolarOne (Qidong) SF220-30-P240 | Hanwha SolarOne (Qidong) SF220-30-P240B | Hanwha SolarOne (Qidong) SF220-30-P240L | Hanwha SolarOne (Qidong) SF220-30-P240L-B | Hanwha SolarOne (Qidong) HSL60M6-HA-0-245T | Hanwha SolarOne (Qidong) HSL60M6-HA-0-245TW | Hanwha SolarOne (Qidong) HSL60M6-HA-4-245T | Hanwha SolarOne (Qidong) HSL60M6-HA-4-245TB | Hanwha SolarOne (Qidong) HSL60M6-HA-4-245TW | Hanwha SolarOne (Qidong) HSL60M6-HB-0-245T | Hanwha SolarOne (Qidong) HSL60M6-HB-0-245TB | Hanwha SolarOne (Qidong) HSL60M6-HB-0-245TW | Hanwha SolarOne (Qidong) HSL60M6-HB-4-245T | Hanwha SolarOne (Qidong) HSL60M6-HB-4-245TB | Hanwha SolarOne (Qidong) HSL60M6-HB-4-245TW | Hanwha Solarone (Qidong) HSL60P6-PA-0-245T | Hanwha SolarOne (Qidong) HSL60P6-PA-0-245TB | Hanwha SolarOne (Qidong) HSL60P6-PA-0-245TW | Hanwha SolarOne (Qidong) HSL60P6-PA-2-245Q | Hanwha SolarOne (Qidong) HSL60P6-PA-2-245QB | Hanwha SolarOne (Qidong) HSL60P6-PA-2-245QW | Hanwha SolarOne (Qidong) HSL60P6-PA-3-245Q | Hanwha SolarOne (Qidong) HSL60P6-PA-3-245QB | Hanwha SolarOne (Qidong) HSL60P6-PA-3-245QW | Hanwha SolarOne (Qidong) HSL60P6-PA-4-245Q | Hanwha SolarOne (Qidong) HSL60P6-PA-4-245QB | Hanwha SolarOne (Qidong) HSL60P6-PA-4-245QW | Hanwha SolarOne (Qidong) HSL60P6-PA-4-245T | Hanwha SolarOne (Qidong) HSL60P6-PA-4-245TB | Hanwha SolarOne (Qidong) HSL60P6-PA-4-245TW | Hanwha Solarone (Qidong) HSL60P6-PB-0-245T | Hanwha SolarOne (Qidong) HSL60P6-PB-0-245TB | Hanwha SolarOne (Qidong) HSL60P6-PB-0-245TW | Hanwha SolarOne (Qidong) HSL60P6-PB-2-245Q | Hanwha SolarOne (Qidong) HSL60P6-PB-2-245QB | Hanwha SolarOne (Qidong) HSL60P6-PB-2-245QW | Hanwha SolarOne (Qidong) HSL60P6-PB-3-245Q | Hanwha SolarOne (Qidong) HSL60P6-PB-3-245QB | Hanwha SolarOne (Qidong) HSL60P6-PB-3-245QW | Hanwha SolarOne (Qidong) HSL60P6-PB-4-245Q | Hanwha SolarOne (Qidong) HSL60P6-PB-4-245QB | Hanwha SolarOne (Qidong) HSL60P6-PB-4-245QW | Hanwha SolarOne (Qidong) HSL60P6-PB-4-245T | Hanwha SolarOne (Qidong) HSL60P6-PB-4-245TB | Hanwha SolarOne (Qidong) HSL60P6-PB-4-245TW | Hanwha SolarOne (Qidong) SF220-30-M245 | Hanwha SolarOne (Qidong) SF220-30-M245B | Hanwha SolarOne (Qidong) SF220-30-M245L | Hanwha SolarOne (Qidong) SF220-30-P245 | Hanwha SolarOne (Qidong) SF220-30-P245B | Hanwha SolarOne (Qidong) SF220-30-P245L | Hanwha SolarOne (Qidong) SF220-30-P245L-B | Hanwha SolarOne (Qidong) HSL60M6-HA-0-250T | Hanwha SolarOne (Qidong) HSL60M6-HA-0-250TW | Hanwha SolarOne (Qidong) HSL60M6-HA-4-250T | Hanwha SolarOne (Qidong) HSL60M6-HA-4-250TB | Hanwha SolarOne (Qidong) HSL60M6-HA-4-250TW | Hanwha SolarOne (Qidong) HSL60M6-HB-0-250T | Hanwha SolarOne (Qidong) HSL60M6-HB-0-250TB | Hanwha SolarOne (Qidong) HSL60M6-HB-0-250TW | Hanwha SolarOne (Qidong) HSL60M6-HB-4-250T | Hanwha SolarOne (Qidong) HSL60M6-HB-4-250TB | Hanwha SolarOne (Qidong) HSL60M6-HB-4-250TW | Hanwha Solarone (Qidong) HSL60P6-PA-0-250T | Hanwha SolarOne (Qidong) HSL60P6-PA-0-250TB | Hanwha SolarOne (Qidong) HSL60P6-PA-0-250TW | Hanwha SolarOne (Qidong) HSL60P6-PA-2-250Q | Hanwha SolarOne (Qidong) HSL60P6-PA-2-250QB | Hanwha SolarOne (Qidong) HSL60P6-PA-2-250QW | Hanwha SolarOne (Qidong) HSL60P6-PA-3-250Q | Hanwha SolarOne (Qidong) HSL60P6-PA-3-250QB | Hanwha SolarOne (Qidong) HSL60P6-PA-3-250QW | Hanwha SolarOne (Qidong) HSL60P6-PA-4-250Q | Hanwha SolarOne (Qidong) HSL60P6-PA-4-250QB | Hanwha SolarOne (Qidong) HSL60P6-PA-4-250QW | Hanwha SolarOne (Qidong) HSL60P6-PA-4-250T | Hanwha SolarOne (Qidong) HSL60P6-PA-4-250TB | Hanwha SolarOne (Qidong) HSL60P6-PA-4-250TW | Hanwha Solarone (Qidong) HSL60P6-PB-0-250T | Hanwha SolarOne (Qidong) HSL60P6-PB-0-250TB | Hanwha SolarOne (Qidong) HSL60P6-PB-0-250TW | Hanwha SolarOne (Qidong) HSL60P6-PB-2-250Q | Hanwha SolarOne (Qidong) HSL60P6-PB-2-250QB | Hanwha SolarOne (Qidong) HSL60P6-PB-2-250QW | Hanwha SolarOne (Qidong) HSL60P6-PB-3-250Q | Hanwha SolarOne (Qidong) HSL60P6-PB-3-250QB | Hanwha SolarOne (Qidong) HSL60P6-PB-3-250QW | Hanwha SolarOne (Qidong) HSL60P6-PB-4-250Q | Hanwha SolarOne (Qidong) HSL60P6-PB-4-250QB | Hanwha SolarOne (Qidong) HSL60P6-PB-4-250QW | Hanwha SolarOne (Qidong) HSL60P6-PB-4-250T | Hanwha SolarOne (Qidong) HSL60P6-PB-4-250TB | Hanwha SolarOne (Qidong) HSL60P6-PB-4-250TW | Hanwha SolarOne (Qidong) HSL60M6-HA-0-255T | Hanwha SolarOne (Qidong) HSL60M6-HA-0-255TW | Hanwha SolarOne (Qidong) HSL60M6-HA-4-255T | Hanwha SolarOne (Qidong) HSL60M6-HA-4-255TB | Hanwha SolarOne (Qidong) HSL60M6-HA-4-255TW | Hanwha SolarOne (Qidong) HSL60M6-HB-0-255T | Hanwha SolarOne (Qidong) HSL60M6-HB-0-255TB | Hanwha SolarOne (Qidong) HSL60M6-HB-0-255TW | Hanwha SolarOne (Qidong) HSL60M6-HB-4-255T | Hanwha SolarOne (Qidong) HSL60M6-HB-4-255TB | Hanwha SolarOne (Qidong) HSL60M6-HB-4-255TW | Hanwha Solarone (Qidong) HSL60P6-PA-0-255T | Hanwha SolarOne (Qidong) HSL60P6-PA-0-255TW | Hanwha SolarOne (Qidong) HSL60P6-PA-4-255T | Hanwha SolarOne (Qidong) HSL60P6-PA-4-255TW | Hanwha Solarone (Qidong) HSL60P6-PB-0-255T | Hanwha SolarOne (Qidong) HSL60P6-PB-0-255TW | Hanwha SolarOne (Qidong) HSL60P6-PB-4-255T | Hanwha SolarOne (Qidong) HSL60P6-PB-4-255TW | Hanwha SolarOne (Qidong) SF260-36-P255 | Hanwha SolarOne (Qidong) SF260-36-P255B | Hanwha SolarOne (Qidong) HSL60M6-HA-0-260T | Hanwha SolarOne (Qidong) HSL60M6-HA-0-260TW | Hanwha SolarOne (Qidong) HSL60M6-HA-4-260T | Hanwha SolarOne (Qidong) HSL60M6-HA-4-260TB | Hanwha SolarOne (Qidong) HSL60M6-HA-4-260TW | Hanwha SolarOne (Qidong) HSL60M6-HB-0-260T | Hanwha SolarOne (Qidong) HSL60M6-HB-0-260TB | Hanwha SolarOne (Qidong) HSL60M6-HB-0-260TW | Hanwha SolarOne (Qidong) HSL60M6-HB-4-260T | Hanwha SolarOne (Qidong) HSL60M6-HB-4-260TB | Hanwha SolarOne (Qidong) HSL60M6-HB-4-260TW | Hanwha SolarOne (Qidong) SF260-36-P260 | Hanwha SolarOne (Qidong) SF260-36-P260B | Hanwha SolarOne (Qidong) SF260-36-P265 | Hanwha SolarOne (Qidong) SF260-36-P265B | Hanwha SolarOne (Qidong) SF260-36-P270 | Hanwha SolarOne (Qidong) SF260-36-P270B | Hanwha SolarOne (Qidong) SF260-36-P270L | Hanwha SolarOne (Qidong) SF260-36-P270L-B | Hanwha Solarone (Qidong) HSL72P6-PA-0-275T | Hanwha SolarOne (Qidong) HSL72P6-PA-0-275TB | Hanwha SolarOne (Qidong) HSL72P6-PA-0-275TW | Hanwha SolarOne (Qidong) HSL72P6-PA-4-275T | Hanwha SolarOne (Qidong) HSL72P6-PA-4-275TB | Hanwha SolarOne (Qidong) HSL72P6-PA-4-275TW | Hanwha SolarOne (Qidong) SF260-36-P275 | Hanwha SolarOne (Qidong) SF260-36-P275B | Hanwha SolarOne (Qidong) SF260-36-P275L | Hanwha SolarOne (Qidong) SF260-36-P275L-B | Hanwha Solarone (Qidong) HSL72P6-PA-0-280T | Hanwha SolarOne (Qidong) HSL72P6-PA-0-280TB | Hanwha SolarOne (Qidong) HSL72P6-PA-0-280TW | Hanwha SolarOne (Qidong) HSL72P6-PA-2-280Q | Hanwha SolarOne (Qidong) HSL72P6-PA-2-280QB | Hanwha SolarOne (Qidong) HSL72P6-PA-2-280QW | Hanwha SolarOne (Qidong) HSL72P6-PA-3-280Q | Hanwha SolarOne (Qidong) HSL72P6-PA-3-280QB | Hanwha SolarOne (Qidong) HSL72P6-PA-3-280QW | Hanwha SolarOne (Qidong) HSL72P6-PA-4-280Q | Hanwha SolarOne (Qidong) HSL72P6-PA-4-280QB | Hanwha SolarOne (Qidong) HSL72P6-PA-4-280QW | Hanwha SolarOne (Qidong) HSL72P6-PA-4-280T | Hanwha SolarOne (Qidong) HSL72P6-PA-4-280TB | Hanwha SolarOne (Qidong) HSL72P6-PA-4-280TW | Hanwha SolarOne (Qidong) HSL72P6-PB-2-280Q | Hanwha SolarOne (Qidong) HSL72P6-PB-2-280QB | Hanwha SolarOne (Qidong) HSL72P6-PB-2-280QW | Hanwha SolarOne (Qidong) HSL72P6-PB-3-280Q | Hanwha SolarOne (Qidong) HSL72P6-PB-3-280QB | Hanwha SolarOne (Qidong) HSL72P6-PB-3-280QW | Hanwha SolarOne (Qidong) HSL72P6-PB-4-280Q | Hanwha SolarOne (Qidong) HSL72P6-PB-4-280QB | Hanwha SolarOne (Qidong) HSL72P6-PB-4-280QW | Hanwha SolarOne (Qidong) SF260-36-P280 | Hanwha SolarOne (Qidong) SF260-36-P280B | Hanwha SolarOne (Qidong) SF260-36-P280L | Hanwha SolarOne (Qidong) SF260-36-P280L-B | Hanwha SolarOne (Qidong) HSL72M6-HA-0-285T | Hanwha SolarOne (Qidong) HSL72M6-HA-0-285TB | Hanwha SolarOne (Qidong) HSL72M6-HA-0-285TW | Hanwha SolarOne (Qidong) HSL72M6-HA-4-285T | Hanwha SolarOne (Qidong) HSL72M6-HA-4-285TB | Hanwha SolarOne (Qidong) HSL72M6-HA-4-285TW | Hanwha SolarOne (Qidong) HSL72M6-HB-0-285T | Hanwha SolarOne (Qidong) HSL72M6-HB-0-285TB | Hanwha SolarOne (Qidong) HSL72M6-HB-0-285TW | Hanwha SolarOne (Qidong) HSL72M6-HB-4-285T | Hanwha SolarOne (Qidong) HSL72M6-HB-4-285TB | Hanwha SolarOne (Qidong) HSL72M6-HB-4-285TW | Hanwha Solarone (Qidong) HSL72P6-PA-0-285T | Hanwha SolarOne (Qidong) HSL72P6-PA-0-285TB | Hanwha SolarOne (Qidong) HSL72P6-PA-0-285TW | Hanwha SolarOne (Qidong) HSL72P6-PA-2-285Q | Hanwha SolarOne (Qidong) HSL72P6-PA-2-285QB | Hanwha SolarOne (Qidong) HSL72P6-PA-2-285QW | Hanwha SolarOne (Qidong) HSL72P6-PA-3-285Q | Hanwha SolarOne (Qidong) HSL72P6-PA-3-285QB | Hanwha SolarOne (Qidong) HSL72P6-PA-3-285QW | Hanwha SolarOne (Qidong) HSL72P6-PA-4-285Q | Hanwha SolarOne (Qidong) HSL72P6-PA-4-285QB | Hanwha SolarOne (Qidong) HSL72P6-PA-4-285QW | Hanwha SolarOne (Qidong) HSL72P6-PA-4-285T | Hanwha SolarOne (Qidong) HSL72P6-PA-4-285TB | Hanwha SolarOne (Qidong) HSL72P6-PA-4-285TW | Hanwha Solarone (Qidong) HSL72P6-PB-0-285T | Hanwha SolarOne (Qidong) HSL72P6-PB-0-285TB | Hanwha SolarOne (Qidong) HSL72P6-PB-0-285TW | Hanwha SolarOne (Qidong) HSL72P6-PB-2-285Q | Hanwha SolarOne (Qidong) HSL72P6-PB-2-285QB | Hanwha SolarOne (Qidong) HSL72P6-PB-2-285QW | Hanwha SolarOne (Qidong) HSL72P6-PB-3-285Q | Hanwha SolarOne (Qidong) HSL72P6-PB-3-285QB | Hanwha SolarOne (Qidong) HSL72P6-PB-3-285QW | Hanwha SolarOne (Qidong) HSL72P6-PB-4-285Q | Hanwha SolarOne (Qidong) HSL72P6-PB-4-285QB | Hanwha SolarOne (Qidong) HSL72P6-PB-4-285QW | Hanwha SolarOne (Qidong) HSL72P6-PB-4-285T | Hanwha SolarOne (Qidong) HSL72P6-PB-4-285TB | Hanwha SolarOne (Qidong) HSL72P6-PB-4-285TW | Hanwha SolarOne (Qidong) SF260-36-P285 | Hanwha SolarOne (Qidong) SF260-36-P285B | Hanwha SolarOne (Qidong) SF260-36-P285L | Hanwha SolarOne (Qidong) SF260-36-P285L-B | Hanwha SolarOne (Qidong) HSL72M6-HA-0-290T | Hanwha SolarOne (Qidong) HSL72M6-HA-0-290TB | Hanwha SolarOne (Qidong) HSL72M6-HA-0-290TW | Hanwha SolarOne (Qidong) HSL72M6-HA-4-290T | Hanwha SolarOne (Qidong) HSL72M6-HA-4-290TB | Hanwha SolarOne (Qidong) HSL72M6-HA-4-290TW | Hanwha SolarOne (Qidong) HSL72M6-HB-0-290T | Hanwha SolarOne (Qidong) HSL72M6-HB-0-290TB | Hanwha SolarOne (Qidong) HSL72M6-HB-0-290TW | Hanwha SolarOne (Qidong) HSL72M6-HB-4-290T | Hanwha SolarOne (Qidong) HSL72M6-HB-4-290TB | Hanwha SolarOne (Qidong) HSL72M6-HB-4-290TW | Hanwha Solarone (Qidong) HSL72P6-PA-0-290T | Hanwha SolarOne (Qidong) HSL72P6-PA-0-290TB | Hanwha SolarOne (Qidong) HSL72P6-PA-0-290TW | Hanwha SolarOne (Qidong) HSL72P6-PA-2-290Q | Hanwha SolarOne (Qidong) HSL72P6-PA-2-290QB | Hanwha SolarOne (Qidong) HSL72P6-PA-2-290QW | Hanwha SolarOne (Qidong) HSL72P6-PA-3-290Q | Hanwha SolarOne (Qidong) HSL72P6-PA-3-290QB | Hanwha SolarOne (Qidong) HSL72P6-PA-3-290QW | Hanwha SolarOne (Qidong) HSL72P6-PA-4-290Q | Hanwha SolarOne (Qidong) HSL72P6-PA-4-290QB | Hanwha SolarOne (Qidong) HSL72P6-PA-4-290QW | Hanwha SolarOne (Qidong) HSL72P6-PA-4-290T | Hanwha SolarOne (Qidong) HSL72P6-PA-4-290TB | Hanwha SolarOne (Qidong) HSL72P6-PA-4-290TW | Hanwha Solarone (Qidong) HSL72P6-PB-0-290T | Hanwha SolarOne (Qidong) HSL72P6-PB-0-290TB | Hanwha SolarOne (Qidong) HSL72P6-PB-0-290TW | Hanwha SolarOne (Qidong) HSL72P6-PB-2-290Q | Hanwha SolarOne (Qidong) HSL72P6-PB-2-290QB | Hanwha SolarOne (Qidong) HSL72P6-PB-2-290QW | Hanwha SolarOne (Qidong) HSL72P6-PB-3-290Q | Hanwha SolarOne (Qidong) HSL72P6-PB-3-290QB | Hanwha SolarOne (Qidong) HSL72P6-PB-3-290QW | Hanwha SolarOne (Qidong) HSL72P6-PB-4-290Q | Hanwha SolarOne (Qidong) HSL72P6-PB-4-290QB | Hanwha SolarOne (Qidong) HSL72P6-PB-4-290QW | Hanwha SolarOne (Qidong) HSL72P6-PB-4-290T | Hanwha SolarOne (Qidong) HSL72P6-PB-4-290TB | Hanwha SolarOne (Qidong) HSL72P6-PB-4-290TW | Hanwha SolarOne (Qidong) SF260-36-P290 | Hanwha SolarOne (Qidong) SF260-36-P290B | Hanwha SolarOne (Qidong) SF260-36-P290L | Hanwha SolarOne (Qidong) SF260-36-P290L-B | Hanwha SolarOne (Qidong) HSL72M6-HA-0-295T | Hanwha SolarOne (Qidong) HSL72M6-HA-0-295TB | Hanwha SolarOne (Qidong) HSL72M6-HA-0-295TW | Hanwha SolarOne (Qidong) HSL72M6-HA-4-295T | Hanwha SolarOne (Qidong) HSL72M6-HA-4-295TB | Hanwha SolarOne (Qidong) HSL72M6-HA-4-295TW | Hanwha SolarOne (Qidong) HSL72M6-HB-0-295T | Hanwha SolarOne (Qidong) HSL72M6-HB-0-295TB | Hanwha SolarOne (Qidong) HSL72M6-HB-0-295TW | Hanwha SolarOne (Qidong) HSL72M6-HB-4-295T | Hanwha SolarOne (Qidong) HSL72M6-HB-4-295TB | Hanwha SolarOne (Qidong) HSL72M6-HB-4-295TW | Hanwha Solarone (Qidong) HSL72P6-PA-0-295T | Hanwha SolarOne (Qidong) HSL72P6-PA-0-295TB | Hanwha SolarOne (Qidong) HSL72P6-PA-0-295TW | Hanwha SolarOne (Qidong) HSL72P6-PA-2-295Q | Hanwha SolarOne (Qidong) HSL72P6-PA-2-295QB | Hanwha SolarOne (Qidong) HSL72P6-PA-2-295QW | Hanwha SolarOne (Qidong) HSL72P6-PA-3-295Q | Hanwha SolarOne (Qidong) HSL72P6-PA-3-295QB | Hanwha SolarOne (Qidong) HSL72P6-PA-3-295QW | Hanwha SolarOne (Qidong) HSL72P6-PA-4-295Q | Hanwha SolarOne (Qidong) HSL72P6-PA-4-295QB | Hanwha SolarOne (Qidong) HSL72P6-PA-4-295QW | Hanwha SolarOne (Qidong) HSL72P6-PA-4-295T | Hanwha SolarOne (Qidong) HSL72P6-PA-4-295TB | Hanwha SolarOne (Qidong) HSL72P6-PA-4-295TW | Hanwha Solarone (Qidong) HSL72P6-PB-0-295T | Hanwha SolarOne (Qidong) HSL72P6-PB-0-295TB | Hanwha SolarOne (Qidong) HSL72P6-PB-0-295TW | Hanwha SolarOne (Qidong) HSL72P6-PB-2-295Q | Hanwha SolarOne (Qidong) HSL72P6-PB-2-295QB | Hanwha SolarOne (Qidong) HSL72P6-PB-2-295QW | Hanwha SolarOne (Qidong) HSL72P6-PB-3-295Q | Hanwha SolarOne (Qidong) HSL72P6-PB-3-295QB | Hanwha SolarOne (Qidong) HSL72P6-PB-3-295QW | Hanwha SolarOne (Qidong) HSL72P6-PB-4-295Q | Hanwha SolarOne (Qidong) HSL72P6-PB-4-295QB | Hanwha SolarOne (Qidong) HSL72P6-PB-4-295QW | Hanwha SolarOne (Qidong) HSL72P6-PB-4-295T | Hanwha SolarOne (Qidong) HSL72P6-PB-4-295TB | Hanwha SolarOne (Qidong) HSL72P6-PB-4-295TW | Hanwha SolarOne (Qidong) SF260-36-P295 | Hanwha SolarOne (Qidong) SF260-36-P295B | Hanwha SolarOne (Qidong) SF260-36-P295L | Hanwha SolarOne (Qidong) SF260-36-P295L-B | Hanwha SolarOne (Qidong) HSL72M6-HA-0-300T | Hanwha SolarOne (Qidong) HSL72M6-HA-0-300TB | Hanwha SolarOne (Qidong) HSL72M6-HA-0-300TW | Hanwha SolarOne (Qidong) HSL72M6-HA-4-300T | Hanwha SolarOne (Qidong) HSL72M6-HA-4-300TB | Hanwha SolarOne (Qidong) HSL72M6-HA-4-300TW | Hanwha SolarOne (Qidong) HSL72M6-HB-0-300T | Hanwha SolarOne (Qidong) HSL72M6-HB-0-300TB | Hanwha SolarOne (Qidong) HSL72M6-HB-0-300TW | Hanwha SolarOne (Qidong) HSL72M6-HB-4-300T | Hanwha SolarOne (Qidong) HSL72M6-HB-4-300TB | Hanwha SolarOne (Qidong) HSL72M6-HB-4-300TW | Hanwha SolarOne (Qidong) HSL72P6-PA-0-300T | Hanwha SolarOne (Qidong) HSL72P6-PA-0-300TW | Hanwha SolarOne (Qidong) HSL72P6-PA-2-300Q | Hanwha SolarOne (Qidong) HSL72P6-PA-2-300QB | Hanwha SolarOne (Qidong) HSL72P6-PA-2-300QW | Hanwha SolarOne (Qidong) HSL72P6-PA-3-300Q | Hanwha SolarOne (Qidong) HSL72P6-PA-3-300QB | Hanwha SolarOne (Qidong) HSL72P6-PA-3-300QW | Hanwha SolarOne (Qidong) HSL72P6-PA-4-300Q | Hanwha SolarOne (Qidong) HSL72P6-PA-4-300QB | Hanwha SolarOne (Qidong) HSL72P6-PA-4-300QW | Hanwha SolarOne (Qidong) HSL72P6-PA-4-300T | Hanwha SolarOne (Qidong) HSL72P6-PA-4-300TW | Hanwha SolarOne (Qidong) HSL72P6-PB-0-300T | Hanwha SolarOne (Qidong) HSL72P6-PB-0-300TW | Hanwha SolarOne (Qidong) HSL72P6-PB-2-300Q | Hanwha SolarOne (Qidong) HSL72P6-PB-2-300QB | Hanwha SolarOne (Qidong) HSL72P6-PB-2-300QW | Hanwha SolarOne (Qidong) HSL72P6-PB-3-300Q | Hanwha SolarOne (Qidong) HSL72P6-PB-3-300QB | Hanwha SolarOne (Qidong) HSL72P6-PB-3-300QW | Hanwha SolarOne (Qidong) HSL72P6-PB-4-300Q | Hanwha SolarOne (Qidong) HSL72P6-PB-4-300QB | Hanwha SolarOne (Qidong) HSL72P6-PB-4-300QW | Hanwha SolarOne (Qidong) HSL72P6-PB-4-300T | Hanwha SolarOne (Qidong) HSL72P6-PB-4-300TW | Hanwha SolarOne (Qidong) HSL72M6-HA-0-305T | Hanwha SolarOne (Qidong) HSL72M6-HA-0-305TB | Hanwha SolarOne (Qidong) HSL72M6-HA-0-305TW | Hanwha SolarOne (Qidong) HSL72M6-HA-4-305T | Hanwha SolarOne (Qidong) HSL72M6-HA-4-305TB | Hanwha SolarOne (Qidong) HSL72M6-HA-4-305TW | Hanwha SolarOne (Qidong) HSL72M6-HB-0-305T | Hanwha SolarOne (Qidong) HSL72M6-HB-0-305TB | Hanwha SolarOne (Qidong) HSL72M6-HB-0-305TW | Hanwha SolarOne (Qidong) HSL72M6-HB-4-305T | Hanwha SolarOne (Qidong) HSL72M6-HB-4-305TB | Hanwha SolarOne (Qidong) HSL72M6-HB-4-305TW | Hanwha SolarOne (Qidong) HSL72P6-PA-2-305Q | Hanwha SolarOne (Qidong) HSL72P6-PA-2-305QB | Hanwha SolarOne (Qidong) HSL72P6-PA-2-305QW | Hanwha SolarOne (Qidong) HSL72P6-PB-2-305Q | Hanwha SolarOne (Qidong) HSL72P6-PB-2-305QB | Hanwha SolarOne (Qidong) HSL72P6-PB-2-305QW | Hanwha SolarOne (Qidong) HSL72M6-HA-0-310T | Hanwha SolarOne (Qidong) HSL72M6-HA-0-310TB | Hanwha SolarOne (Qidong) HSL72M6-HA-0-310TW | Hanwha SolarOne (Qidong) HSL72M6-HA-4-310T | Hanwha SolarOne (Qidong) HSL72M6-HA-4-310TB | Hanwha SolarOne (Qidong) HSL72M6-HA-4-310TW | Hanwha SolarOne (Qidong) HSL72M6-HB-0-310T | Hanwha SolarOne (Qidong) HSL72M6-HB-0-310TB | Hanwha SolarOne (Qidong) HSL72M6-HB-0-310TW | Hanwha SolarOne (Qidong) HSL72M6-HB-4-310T | Hanwha SolarOne (Qidong) HSL72M6-HB-4-310TB | Hanwha SolarOne (Qidong) HSL72M6-HB-4-310TW | Hanwha SolarOne Hong Kong HSL60P-PA-0-235K | Hanwha SolarOne Hong Kong HSL60P-PA-0-240K | Hanwha SolarOne Hong Kong HSL60P-PA-0-245K | Hanwha SolarOne Hong Kong HSL60P-PA-0-250K | Hanwha SolarOne Hong Kong HSL72P-PA-0-280K | Hanwha SolarOne Hong Kong HSL72P-PA-0-285K | Hanwha SolarOne Hong Kong HSL72P-PA-0-290K | Hanwha SolarOne Hong Kong HSL72P-PA-0-295K | HC Solar Power HCP175D-24 | HC Solar Power HCP180D-24 | HC Solar Power HCP185D-24 | HC Solar Power HCP190D-24 | HC Solar Power HCP195D-24 | HC Solar Power HCP230P-20 | HC Solar Power HCP235P-20 | HC Solar Power HCP240P-20 | HC Solar Power HCP245P-24 | HC Solar Power HCP250P-24 | HC Solar Power HCP255P-24 | HC Solar Power HCP260P-24 | HC Solar Power HCP265P-24 | HC Solar Power HCP270P-24 | HC Solar Power HCP275P-24 | HC Solar Power HCP280P-24 | Heliene 60P215 | Heliene 60P220 | Heliene 60P225 | Heliene 60M230 | Heliene 60P230 | Heliene 60M235 | Heliene 60M240 | Heliene 60M245 | Heliene 60M250 | Heliene 60M255 | Heliene 60M260 | Heliene 72P260 | Heliene 60M265 | Heliene 72P265 | Heliene 72P270 | Heliene 72P275 | Heliene 72M280 | Heliene 72M285 | Heliene 72M290 | Heliene 72M295 | Heliene 72M300 | Heliene 72M305 | Heliene 72M310 | Heliene 72M315 | Heliene 96M390 | Heliene 96M395 | Heliene 96M400 | Heliene 96M405 | Heliene 96M410 | Heliene 96M415 | Heliene 96M420 | Helios Energy Europe HEE210UA62 | Helios Energy Europe HEE210UA63 | Helios Energy Europe HEE210U | Helios Energy Europe HEE210UA64 | Helios Energy Europe HEE210UA65 | Helios Energy Europe HEE215MA64 | Helios Energy Europe HEE215MA65 | Helios Energy Europe HEE215M | Helios Energy Europe HEE215MA66 | Helios Energy Europe HEE215MA67 | Helios Energy Europe 60M250 | Helios Energy Europe HEE215MA68 | Helios Energy Europe 60M255 | Helios Energy Europe 60M260 | Helios Energy Europe HEE275AU72 | Helios Energy Europe 60M265 | Helios Energy Europe HEE275AU73 | Helios Energy Europe HEE275AU74 | Helios Energy Europe HEE275U | Helios Energy Europe HEE275AU75 | Helios Energy Europe HEE300MA74 | Helios Energy Europe HEE300MA75 | Helios Energy Europe HEE300M | Helios Energy Europe HEE300MA76 | Helios Energy Europe HEE300MA77 | Helios Energy Europe HEE300MA78 | Helios Energy Europe 72M305 | Helios Energy Europe 72M310 | Helios Energy Europe 72M315 | Helios Energy Europe 96M390 | Helios Energy Europe 96M395 | Helios Energy Europe 96M400 | Helios Energy Europe 96M405 | Helios Energy Europe 96M410 | Helios Energy Europe 96M415 | Helios Energy Europe 96M420 | Helios USA 6T p215 | Helios USA 6T p220 | Helios USA 6T p225 | Helios USA 6T 230 | Helios USA 6T p230 | Helios USA 6T 235 | Helios USA 6T 240 | Helios USA 6T 245 | Helios USA 6T 250 | Helios USA 6T 255 | Helios USA 6TA | Helios USA 6T 260 | Helios USA 6T 265 | Helios USA 7T2 280 | Helios USA 7T2 285 | Helios USA 7T2 290 | Helios USA 7T2 295 | Helios USA 7T2 300 | Helios USA 7T2 305 | Helios USA 7T2 310 | Helios USA 7T2 315 | Helios USA 9T6 390 | Helios USA 9T6 395 | Helios USA 9T6 400 | Helios USA 9T6 405 | Helios USA 9T6 410 | Helios USA 9T6 415 | Helios USA 9T6 420 | HelioVolt HVC-170X | HelioVolt HVC-190X | Hengdian Group DMEGC Magnetics DM175-M125-72 | Hengdian Group DMEGC Magnetics DM180-M125-72 | Hengdian Group DMEGC Magnetics DM185-M125-72 | Hengdian Group DMEGC Magnetics DM190-M125-72 | Hengdian Group DMEGC Magnetics DM195-M125-72 | Hengdian Group DMEGC Magnetics DM210-P156-60 | Hengdian Group DMEGC Magnetics DM215-P156-60 | Hengdian Group DMEGC Magnetics DM220-P156-60 | Hengdian Group DMEGC Magnetics DM225-P156-60 | Hengdian Group DMEGC Magnetics DM230-M156-60 | Hengdian Group DMEGC Magnetics DM230-P156-60 | Hengdian Group DMEGC Magnetics DM235-M156-60 | Hengdian Group DMEGC Magnetics DM235-P156-60 | Hengdian Group DMEGC Magnetics DM240-M156-60 | Hengdian Group DMEGC Magnetics DM240-P156-60 | Hengdian Group DMEGC Magnetics DM245-M156-60 | Hengdian Group DMEGC Magnetics DM245-P156-60 | Hengdian Group DMEGC Magnetics DM250-M156-60 | Hengdian Group DMEGC Magnetics DM250-P156-60 | Hengdian Group DMEGC Magnetics DM250-P156-72 | Hengdian Group DMEGC Magnetics DM255-P156-60 | Hengdian Group DMEGC Magnetics DM255-P156-72 | Hengdian Group DMEGC Magnetics DM260-P156-60 | Hengdian Group DMEGC Magnetics DM260-P156-72 | Hengdian Group DMEGC Magnetics DM265-M156-72 | Hengdian Group DMEGC Magnetics DM265-P156-72 | Hengdian Group DMEGC Magnetics DM270-M156-72 | Hengdian Group DMEGC Magnetics DM270-P156-72 | Hengdian Group DMEGC Magnetics DM275-M156-72 | Hengdian Group DMEGC Magnetics DM275-P156-72 | Hengdian Group DMEGC Magnetics DM280-M156-72 | Hengdian Group DMEGC Magnetics DM280-P156-72 | Hengdian Group DMEGC Magnetics DM285-M156-72 | Hengdian Group DMEGC Magnetics DM285-P156-72 | Hengdian Group DMEGC Magnetics DM290-M156-72 | Hengdian Group DMEGC Magnetics DM290-P156-72 | Hengdian Group DMEGC Magnetics DM295-M156-72 | Hengdian Group DMEGC Magnetics DM295-P156-72 | Hengdian Group DMEGC Magnetics DM300-P156-72 | Hengdian Group DMEGC Magnetics DM305-P156-72 | Hengji PV-Tech Energy HJM085M-12 | Hengji PV-Tech Energy HJM090M-12 | Hengji PV-Tech Energy HJM095M-12 | Hengji PV-Tech Energy HJM170M-24 | Hengji PV-Tech Energy HJM175M-24 | Hengji PV-Tech Energy HJM180M-24 | Hengji PV-Tech Energy HJM180P-16 | Hengji PV-Tech Energy HJM185M-24 | Hengji PV-Tech Energy HJM190M-24 | Hengji PV-Tech Energy HJM190M-28 | Hengji PV-Tech Energy HJM190P-16 | Hengji PV-Tech Energy HJM200M-28 | Hengji PV-Tech Energy HJM200P-16 | Hengji PV-Tech Energy HJM200P-18 | Hengji PV-Tech Energy HJM210M-28 | Hengji PV-Tech Energy HJM210P-18 | Hengji PV-Tech Energy HJM220M-28 | Hengji PV-Tech Energy HJM220P-18 | Hengji PV-Tech Energy HJM230M-28 | Hengji PV-Tech Energy HJM230P-20 | Hengji PV-Tech Energy HJM240P-20 | Hengji PV-Tech Energy HJM250P-20 | Hengji PV-Tech Energy HJM270P-24 | Hengji PV-Tech Energy HJM280P-24 | Hengji PV-Tech Energy HJM290P-24 | HHV Solar Technologies HSTUBC12095P | HHV Solar Technologies HSTUBC12100P | HHV Solar Technologies HSTUBC12105P | HHV Solar Technologies HSTUBF12130P | HHV Solar Technologies HSTUAF12135M | HHV Solar Technologies HSTUBF12135P | HHV Solar Technologies HSTUAF12140M | HHV Solar Technologies HSTUBF12140P | HHV Solar Technologies HSTUAF12145M | HHV Solar Technologies HSTUBF12175P | HHV Solar Technologies HSTUAF12180M | HHV Solar Technologies HSTUBF12180P | HHV Solar Technologies HSTUAF12185M | HHV Solar Technologies HSTUBF12185P | HHV Solar Technologies HSTUAF12190M | HHV Solar Technologies HSTUBF12190P | HHV Solar Technologies HSTUAF12195M | HHV Solar Technologies HSTUBF12195P | HHV Solar Technologies HSTUBF12200P | HHV Solar Technologies HSTUAF12205M | HHV Solar Technologies HSTUBF12205P | HHV Solar Technologies HSTUAF12210M | HHV Solar Technologies HSTUBF12210P | HHV Solar Technologies HSTUAF12215M | HHV Solar Technologies HSTUBF24215P | HHV Solar Technologies HSTUCF24215P | HHV Solar Technologies HSTUAF12220M | HHV Solar Technologies HSTUBF24220P | HHV Solar Technologies HSTUCF24220P | HHV Solar Technologies HSTUAF24225M | HHV Solar Technologies HSTUBF24225P | HHV Solar Technologies HSTUCF24225P | HHV Solar Technologies HSTUAF24230M | HHV Solar Technologies HSTUBF24230P | HHV Solar Technologies HSTUCF24230P | HHV Solar Technologies HSTUAF24235M | HHV Solar Technologies HSTUBF24235P | HHV Solar Technologies HSTUCF24235P | HHV Solar Technologies HSTUAF24240M | HHV Solar Technologies HSTUAF24245M | HHV Solar Technologies HSTUAF24260M | HHV Solar Technologies HSTUBF24260P | HHV Solar Technologies HSTUCF24260P | HHV Solar Technologies HSTUAF24265M | HHV Solar Technologies HSTUBF24265P | HHV Solar Technologies HSTUCF24265P | HHV Solar Technologies HSTUAF24270M | HHV Solar Technologies HSTUBF24270P | HHV Solar Technologies HSTUCF24270P | HHV Solar Technologies HSTUAF24275M | HHV Solar Technologies HSTUBF24275P | HHV Solar Technologies HSTUCF24275P | HHV Solar Technologies HSTUAF24280M | HHV Solar Technologies HSTUBF24280P | HHV Solar Technologies HSTUCF24280P | HHV Solar Technologies HSTUAF24285M | HHV Solar Technologies HSTUAF24290M | HHV Solar Technologies HSTUAF24295M | Himin Clean Energy Holdings HG-160S | Himin Clean Energy Holdings HG-165S | Himin Clean Energy Holdings HG-170S | Himin Clean Energy Holdings HG-175S | Himin Clean Energy Holdings HG-180S | Himin Clean Energy Holdings HG-185S | Honda Soltec HEM120PUB | Honda Soltec HEM125PUB | Honda Soltec HEM130PUB | Hunan Sunzone Optoelectronics Energy SZ180M-36 | Hunan Sunzone Optoelectronics Energy SZ185M-36 | Hunan Sunzone Optoelectronics Energy SZ190M-36 | Hunan Sunzone Optoelectronics Energy SZ220P-29 | Hunan Sunzone Optoelectronics Energy SZ225P-29 | Hunan Sunzone Optoelectronics Energy SZ230P-29 | Hunan Sunzone Optoelectronics Energy SZ235P-29 | Hunan Sunzone Optoelectronics Energy SZ240P-29 | Hunan Sunzone Optoelectronics Energy SZ275P-35 | Hunan Sunzone Optoelectronics Energy SZ280P-35 | Hunan Sunzone Optoelectronics Energy SZ285P-35 | Hunan Sunzone Optoelectronics Energy SZ290P-35 | Hyundai Heavy Industries HiS-M191SF | Hyundai Heavy Industries HiS-M194SF | Hyundai Heavy Industries HiS-M197SF | Hyundai Heavy Industries HiS-M200SF | Hyundai Heavy Industries HiS-M203SF | Hyundai Heavy Industries HiS-M206SF | Hyundai Heavy Industries HiS-S206SF | Hyundai Heavy Industries HiS-M209SF | Hyundai Heavy Industries HiS-S209SF | Hyundai Heavy Industries HiS-M212SF | Hyundai Heavy Industries HiS-M212SG | Hyundai Heavy Industries HiS-S212SF | Hyundai Heavy Industries HiS-M215SF | Hyundai Heavy Industries HiS-M215SG | Hyundai Heavy Industries HiS-S215SF | Hyundai Heavy Industries HiS-M218SG | Hyundai Heavy Industries HiS-S218SF | Hyundai Heavy Industries HiS-M221SG | Hyundai Heavy Industries HiS-S221SF | Hyundai Heavy Industries HiS-M223MG | Hyundai Heavy Industries HiS-M223MG(BK) | Hyundai Heavy Industries HiS-M224SG | Hyundai Heavy Industries HiS-S224SF | Hyundai Heavy Industries HiS-S224SG | Hyundai Heavy Industries HiS-M225MG | Hyundai Heavy Industries HiS-M225MG(BK) | Hyundai Heavy Industries HiS-M227SG | Hyundai Heavy Industries HiS-S227SG | Hyundai Heavy Industries HiS-M228MG | Hyundai Heavy Industries HiS-M228MG(BK) | Hyundai Heavy Industries HiS-M230MG | Hyundai Heavy Industries HiS-M230MG(BK) | Hyundai Heavy Industries HiS-M230SG | Hyundai Heavy Industries HiS-S230SG | Hyundai Heavy Industries HiS-M233MG | Hyundai Heavy Industries HiS-M233MG(BK) | Hyundai Heavy Industries HiS-M233SG | Hyundai Heavy Industries HiS-S233MG | Hyundai Heavy Industries HiS-S233MG(BK) | Hyundai Heavy Industries HiS-S233SG | Hyundai Heavy Industries HiS-M235MG | Hyundai Heavy Industries HiS-M235MG(BK) | Hyundai Heavy Industries HiS-S235MG | Hyundai Heavy Industries HiS-S235MG(BK) | Hyundai Heavy Industries HiS-M236SG | Hyundai Heavy Industries HiS-S236SG | Hyundai Heavy Industries HiS-M238MG | Hyundai Heavy Industries HiS-M238MG(BK) | Hyundai Heavy Industries HiS-S238MG | Hyundai Heavy Industries HiS-S238MG(BK) | Hyundai Heavy Industries HiS-M239SG | Hyundai Heavy Industries HiS-S239SG | Hyundai Heavy Industries HiS-M240MG | Hyundai Heavy Industries HiS-M240MG(BK) | Hyundai Heavy Industries HiS-S240MG | Hyundai Heavy Industries HiS-S240MG(BK) | Hyundai Heavy Industries HiS-M242SG | Hyundai Heavy Industries HiS-S242SG | Hyundai Heavy Industries HiS-M243MG | Hyundai Heavy Industries HiS-M243MG(BK) | Hyundai Heavy Industries HiS-S243MG | Hyundai Heavy Industries HiS-S243MG(BK) | Hyundai Heavy Industries HiS-M245MG | Hyundai Heavy Industries HiS-M245MG(BK) | Hyundai Heavy Industries HiS-S245MG | Hyundai Heavy Industries HiS-S245MG(BK) | Hyundai Heavy Industries HiS-M248MG | Hyundai Heavy Industries HiS-M248MG(BK) | Hyundai Heavy Industries HiS-S248MG | Hyundai Heavy Industries HiS-S248MG(BK) | Hyundai Heavy Industries HiS-M250MG | Hyundai Heavy Industries HiS-M250MG(BK) | Hyundai Heavy Industries HiS-S250MG | Hyundai Heavy Industries HiS-S250MG(BK) | Hyundai Heavy Industries HiS-M253MG(BK) | Hyundai Heavy Industries HiS-S253MG | Hyundai Heavy Industries HiS-S253MG(BK) | Hyundai Heavy Industries HiS-M255MG(BK) | Hyundai Heavy Industries HiS-S255MG | Hyundai Heavy Industries HiS-S255MG(BK) | Hyundai Heavy Industries HiS-S258MG | Hyundai Heavy Industries HiS-S260MG | Hyundai Heavy Industries HiS-S263MG | Hyundai Heavy Industries HiS-S265MG | Hyundai Heavy Industries HiS-S268MG | Hyundai Heavy Industries HiS-S270MG | Hyundai Heavy Industries HiS-M273MI | Hyundai Heavy Industries HiS-S273MG | Hyundai Heavy Industries HiS-M275MI | Hyundai Heavy Industries HiS-S275MG | Hyundai Heavy Industries HiS-M278MI | Hyundai Heavy Industries HiS-M280MI | Hyundai Heavy Industries HiS-S280MI | Hyundai Heavy Industries HiS-M283MI | Hyundai Heavy Industries HiS-S283MI | Hyundai Heavy Industries HiS-M285MI | Hyundai Heavy Industries HiS-S285MI | Hyundai Heavy Industries HiS-M288MI | Hyundai Heavy Industries HiS-S288MI | Hyundai Heavy Industries HiS-M290MI | Hyundai Heavy Industries HiS-S290MI | Hyundai Heavy Industries HiS-M293MI | Hyundai Heavy Industries HiS-S293MI | Hyundai Heavy Industries HiS-M295MI | Hyundai Heavy Industries HiS-S295MI | Hyundai Heavy Industries HiS-M298MI | Hyundai Heavy Industries HiS-S298MI | Hyundai Heavy Industries HiS-M300MI | Hyundai Heavy Industries HiS-S300MI | Hyundai Heavy Industries HiS-S303MI | Hyundai Heavy Industries HiS-S305MI | Innotech Solar ITS210XXXX | Innotech Solar ITS220Eyz2 | Innotech Solar ITS220Fyz2 | Innotech Solar ITS220Myz2 | Innotech Solar ITS220Nyz2 | Innotech Solar ITS215XXXX | Innotech Solar ITS220Eyz3 | Innotech Solar ITS220Fyz3 | Innotech Solar ITS220Myz3 | Innotech Solar ITS220Nyz3 | Innotech Solar x220 | Innotech Solar ITS225XXXX | Innotech Solar x225 | Innotech Solar ITS220Eyz4 | Innotech Solar ITS220Fyz4 | Innotech Solar ITS220Mxy4 | Innotech Solar ITS220Nxy4 | Innotech Solar ITS230XXXX | Innotech Solar x230 | Innotech Solar x235 | Innotech Solar x240 | Innotech Solar x245 | Innotech Solar ITS270Eyz1 | Innotech Solar ITS270Fyz1 | Innotech Solar ITS270Myz1 | Innotech Solar ITS270Nyz1 | Innotech Solar x250 | Innotech Solar x255 | Innotech Solar ITS270Eyz2 | Innotech Solar ITS270Fyz2 | Innotech Solar ITS270Myz2 | Innotech Solar ITS270Nyz2 | Innotech Solar x260 | Innotech Solar x265 | Innotech Solar ITS270Eyz3 | Innotech Solar ITS270Fyz3 | Innotech Solar ITS270Myz3 | Innotech Solar ITS270Nyz3 | Innovosolar International TEM165M | Innovosolar International TEM170M | Innovosolar International TEM175M | Innovosolar International TEM180M | Instalaciones Pevafersa IP-VA180 | Instalaciones Pevafersa IP-VAP210 | Instalaciones Pevafersa IP-220 GG | Instalaciones Pevafersa IP-225 GG | Instalaciones Pevafersa IP-230 GG | Instalaciones Pevafersa IP-VAP230 | Instalaciones Pevafersa IP-235 GG | Integrated Power IPC175M01 | Integrated Power IPC175M01-US | Integrated Power IPC175P01 | Integrated Power IPC175P01-US | Integrated Power IPC180M01 | Integrated Power IPC180M01-US | Integrated Power IPC180P01 | Integrated Power IPC180P01-US | Integrated Power IPC185M01 | Integrated Power IPC185M01-US | Integrated Power IPC185P01 | Integrated Power IPC185P01-US | Integrated Power IPC190P01 | Integrated Power IPC190P01-US | Integrated Power IPC200P01 | Integrated Power IPC200P01-US | Integrated Power IPC205P01 | Integrated Power IPC205P01-US | Integrated Power IPC210P01 | Integrated Power IPC210P01-US | Integrated Power IPC215P01 | Integrated Power IPC215P01-US | Integrated Power IPC220P01 | Integrated Power IPC220P01-US | Integrated Power IPC225P01 | Integrated Power IPC225P01-US | Integrated Power IPC230P01 | Integrated Power IPC230P01-US | Integrated Power IPC235P01 | Integrated Power IPC235P01-US | Integrated Power IPC240P01 | Integrated Power IPC240P01-US | Integrated Power IPC245P01 | Integrated Power IPC245P01-US | Integrated Power IPC250P01 | Integrated Power IPC250P01-US | Integrated Power IPC255P01 | Integrated Power IPC255P01-US | Integrated Power IPC260P01 | Integrated Power IPC260P01-US | Integrated Power IPC265P01 | Integrated Power IPC265P01-US | Integrated Power IPC270P01 | Integrated Power IPC270P01-US | Integrated Power IPC275P01 | Integrated Power IPC275P01-US | Integrated Power IPC280P01 | Integrated Power IPC280P01-US | Inventec Energy IECS-6P66-125 | Inventec Energy IECS-6M66-130 | Inventec Energy IECS-6P66-130 | Inventec Energy IECS-6M66-135 | Inventec Energy IECS-6P66-135 | Inventec Energy IECS-6M66-140 | Inventec Energy IECS-6P66-140 | Inventec Energy IECS-6M66-145 | Inventec Energy IECS-6P66-145 | Inventec Energy IECS-6P67-145 | Inventec Energy IECS-6M66-150 | Inventec Energy IECS-6M67-150 | Inventec Energy IECS-6P67-150 | Inventec Energy IECS-6M67-155 | Inventec Energy IECS-6P67-155 | Inventec Energy IECS-6M67-160 | Inventec Energy IECS-6P67-160 | Inventec Energy IECS-6M67-165 | Inventec Energy IECS-6P67-165 | Inventec Energy IECS-6P68-165 | Inventec Energy IECS-6M67-170 | Inventec Energy IECS-6M68-170 | Inventec Energy IECS-6P67-170 | Inventec Energy IECS-6P68-170 | Inventec Energy IECS-6M67-175 | Inventec Energy IECS-6M68-175 | Inventec Energy IECS-6P67-175 | Inventec Energy IECS-6P68-175 | Inventec Energy IECS-6M68-180 | Inventec Energy IECS-6M68-185 | Inventec Energy IECS-6P68-185 | Inventec Energy IECS-6M68-190 | 